simulink model "hrg_wa_v8_calibrated"  (R2025a)
settings: Solver=ode4  StartTime=0.0  StopTime=wl_stop  FixedStep=wl_Tp  RelTol=1e-3
PostLoadFcn:
  | addpath(fileparts(fileparts(get_param('hrg_wa_v8_calibrated','FileName')))); w8_setup(getVariable(get_param('hrg_wa_v8_calibrated','ModelWorkspace'),'v8_saved_configuration'));
model workspace (MAT data in the model file):
  v7_saved_configuration.stage = 5
  v7_saved_configuration.name = 'hrg_wa_v8_calibrated'
  v7_saved_configuration.head.sourceProfile = 'C:\Users\11725\Desktop\HRG_WA\HRG_WA_Digital_ASIC_MATLAB_v4_6_5_FRP_validation_fix\HRG_WA\config\head_default.json'
  v7_saved_configuration.head.measurementStatus = 'assumed, not a measured head'
  v7_saved_configuration.head.f0 = 5000
  v7_saved_configuration.head.Q = 2000000
  v7_saved_configuration.head.bryan = 0.277
  v7_saved_configuration.head.gamma = 0.00785398163397
  v7_saved_configuration.head.dgamma = 0
  v7_saved_configuration.head.dampingAxis = 0.296705972839
  v7_saved_configuration.head.splitHz = 0
  v7_saved_configuration.head.stiffnessAxis = 0.715584993318
  v7_saved_configuration.head.detuningHz = 0
  v7_saved_configuration.head.duffingHz = 0
  v7_saved_configuration.head.temperatureCoeff = -1.8e-05
  v7_saved_configuration.head.referenceTemperature = 25
  v7_saved_configuration.head.detect = [1.012  0; 0  0.989]
  v7_saved_configuration.head.detectPhase = [0; 0]
  v7_saved_configuration.head.drive = [1  0; 0  1]
  v7_saved_configuration.head.detectCubic = 0
  v7_saved_configuration.head.iqBits = 0
  v7_saved_configuration.head.iqFullScale = 2
  v7_saved_configuration.head.energyTarget = 1
  v7_saved_configuration.head.initialEnergy = 1
  v7_saved_configuration.head.initialTheta = 0.13962634016
  v7_saved_configuration.head.initialQuadRatio = 0
  v7_saved_configuration.head.energyKp = 4.02123859659
  v7_saved_configuration.head.energyKi = 12.6330936334
  v7_saved_configuration.head.quadKp = 6.03185789489
  v7_saved_configuration.head.quadKi = 28.4244606751
  v7_saved_configuration.head.pllKp = 1.28
  v7_saved_configuration.head.pllKi = 4.02123859659
  v7_saved_configuration.head.energyLimit = 20
  v7_saved_configuration.head.quadLimit = 2
  v7_saved_configuration.head.pllLimitHz = 2
  v7_saved_configuration.head.antiWindup = 5
  v7_saved_configuration.head.loopEnable = 1
  v7_saved_configuration.head.Ts = 0.001
  v7_saved_configuration.head.rateTau = 0.00353677651315
  v7_saved_configuration.head.energyThreshold = 0.02
  v7_saved_configuration.head.angleThreshold = 0.01
  v7_saved_configuration.head.duration = 12
  v7_saved_configuration.head.omega = 1.3962634016
  v7_saved_configuration.head.virtualRate = 0
  v7_saved_configuration.head.temperature = 25
  v7_saved_configuration.head.fullStep = 2e-06
  v7_saved_configuration.fsAdc = 40000
  v7_saved_configuration.fsPlant = 800000
  v7_saved_configuration.duration = 2
  v7_saved_configuration.seed = 20261021
  v7_saved_configuration.massKg = 1e-06
  v7_saved_configuration.displacementM = 4e-07
  v7_saved_configuration.gapM = 5e-06
  v7_saved_configuration.c0F = 1e-12
  v7_saved_configuration.cfF = 1e-12
  v7_saved_configuration.rfOhm = 1000000000
  v7_saved_configuration.biasV = 10
  v7_saved_configuration.cvBandwidthHz = 30000
  v7_saved_configuration.pgaBandwidthHz = 30000
  v7_saved_configuration.pgaGain = 1
  v7_saved_configuration.cvEnVrtHz = 1e-08
  v7_saved_configuration.cvInArtHz = 1e-14
  v7_saved_configuration.temperatureK = 298.15
  v7_saved_configuration.pgaNoiseVrtHz = 1e-08
  v7_saved_configuration.afeOffsetV = [0; 0]
  v7_saved_configuration.afeLimitV = 1.8
  v7_saved_configuration.adcBits = 18
  v7_saved_configuration.adcFsV = 2
  v7_saved_configuration.adcOffsetV = [0; 0]
  v7_saved_configuration.adcGain = [1; 1]
  v7_saved_configuration.adcInlCubic = 0
  v7_saved_configuration.jitterRmsS = 2e-09
  v7_saved_configuration.channelSkewS = 0
  v7_saved_configuration.adcDelay = 1
  v7_saved_configuration.adcArchitecture = 'nyquist'
  v7_saved_configuration.cicStages = 3
  v7_saved_configuration.fir = [0.111111111111 0.222222222222 0.333333333333 0.222222222222 0.111111111111]
  v7_saved_configuration.dacBits = 16
  v7_saved_configuration.dacFsV = 2
  v7_saved_configuration.dacDelay = 1
  v7_saved_configuration.dacInlCubic = 0
  v7_saved_configuration.dacArchitecture = 'nyquist'
  v7_saved_configuration.driveNPerV = 1e-07
  v7_saved_configuration.driverBandwidthHz = 50000
  v7_saved_configuration.driverGain = [1.018; 0.982]
  v7_saved_configuration.driverSlewVPerS = 200000
  v7_saved_configuration.driverNoiseVrtHz = 2e-08
  v7_saved_configuration.driverLimitV = 1.8
  v7_saved_configuration.feedthroughF = 0
  v7_saved_configuration.pipelineCtrl = 3
  v7_saved_configuration.iqFractionBits = 22
  v7_saved_configuration.controlFractionBits = 22
  v7_saved_configuration.antiAliasHz = 18000
  v7_saved_configuration.noiseEnable = 0
  v7_saved_configuration.circuitEnable = 1
  v7_saved_configuration.kalman = 1
  v7_saved_configuration.online = 0
  v7_saved_configuration.frp = 0
  v7_saved_configuration.calibrationPermit = 0
  v7_saved_configuration.frpSequence = 0
  v7_saved_configuration.frpFreeze = 0
  v7_saved_configuration.frpTheta = [0; 0; 0; 0; 0; 0; 0; 0; 0]
  v7_saved_configuration.matrixApply = 0
  v7_saved_configuration.compensationApply = 0
  v7_saved_configuration.temperatureCompensate = 0
  v7_saved_configuration.temperatureBiasCoefficients = [0; 0; 0]
  v7_saved_configuration.zeroRateCertified = 0
  v7_saved_configuration.virtualRate = 0
  v7_saved_configuration.inputRate = 1.3962634016
  v7_saved_configuration.inputFrequencyHz = 0
  v7_saved_configuration.inputRateAmplitude = 0
  v7_saved_configuration.temperatureC = 25
  v7_saved_configuration.temperatureRampCPerS = 0
  v7_saved_configuration.observers = 1
  v7_saved_configuration.spectra = 1
  v7_saved_configuration.maxLogPoints = 1600001
  v7_saved_configuration.sdmLeak = 0.9999
  v7_saved_configuration.sdmReferenceV = 2
  v7_saved_configuration.tdmEnable = 0
  v7_saved_configuration.knownPhaseCalibrationRad = 0
  v7_saved_configuration.virtualGainCalibration = 1
  v7_saved_configuration.learnStartS = 0.25
  v7_saved_configuration.measurementStatus = 'unmeasured research assumptions; replace with measured head and interface data'
  v7_saved_configuration.scope = 'Behavioral circuit interfaces, not transistor or bit-true RTL signoff'
  v7_saved_configuration.v7.schemaVersion = 1
  v7_saved_configuration.v7.status = 'unmeasured research assumptions; replace with measured head and interface data'
  v7_saved_configuration.v7.mechanicalProfile = 'HRG_WA_Digital_ASIC_MATLAB_v4_6_5_FRP_validation_fix/HRG_WA/config/head_default.json'
  v7_saved_configuration.v7.headSimulation.Ts = 0.001
  v7_saved_configuration.v7.headSimulation.initialEnergy = 1
  v7_saved_configuration.v7.headSimulation.initialQuadRatio = 0
  v7_saved_configuration.v7.headSimulation.rateTau = 0.00353677651315
  v7_saved_configuration.v7.circuit.fsAdc = 40000
  v7_saved_configuration.v7.circuit.massKg = 1e-06
  v7_saved_configuration.v7.circuit.displacementM = 1e-07
  v7_saved_configuration.v7.circuit.gapM = 5e-06
  v7_saved_configuration.v7.circuit.c0F = 1e-12
  v7_saved_configuration.v7.circuit.biasV = 10
  v7_saved_configuration.v7.circuit.cvBandwidthHz = 30000
  v7_saved_configuration.v7.circuit.pgaBandwidthHz = 30000
  v7_saved_configuration.v7.circuit.cvEnVrtHz = 1e-08
  v7_saved_configuration.v7.circuit.cvInArtHz = 1e-14
  v7_saved_configuration.v7.circuit.temperatureK = 298.15
  v7_saved_configuration.v7.circuit.pgaNoiseVrtHz = 1e-08
  v7_saved_configuration.v7.circuit.afeOffsetV = [0; 0]
  v7_saved_configuration.v7.circuit.afeLimitV = 1.8
  v7_saved_configuration.v7.circuit.adcBits = 18
  v7_saved_configuration.v7.circuit.adcFsV = 2
  v7_saved_configuration.v7.circuit.adcOffsetV = [0; 0]
  v7_saved_configuration.v7.circuit.adcGain = [1; 1]
  v7_saved_configuration.v7.circuit.adcInlCubic = 0
  v7_saved_configuration.v7.circuit.jitterRmsS = 2e-09
  v7_saved_configuration.v7.circuit.channelSkewS = 0
  v7_saved_configuration.v7.circuit.adcDelay = 1
  v7_saved_configuration.v7.circuit.adcArchitecture = 'nyquist'
  v7_saved_configuration.v7.circuit.cicStages = 3
  v7_saved_configuration.v7.circuit.fir = [0.111111111111; 0.222222222222; 0.333333333333; 0.222222222222; 0.111111111111]
  v7_saved_configuration.v7.circuit.dacBits = 16
  v7_saved_configuration.v7.circuit.dacFsV = 2
  v7_saved_configuration.v7.circuit.dacDelay = 1
  v7_saved_configuration.v7.circuit.dacInlCubic = 0
  v7_saved_configuration.v7.circuit.dacArchitecture = 'nyquist'
  v7_saved_configuration.v7.circuit.driveNPerV = 1e-07
  v7_saved_configuration.v7.circuit.driverBandwidthHz = 50000
  v7_saved_configuration.v7.circuit.driverGain = [1; 1]
  v7_saved_configuration.v7.circuit.driverSlewVPerS = 200000
  v7_saved_configuration.v7.circuit.driverNoiseVrtHz = 2e-08
  v7_saved_configuration.v7.circuit.driverLimitV = 1.8
  v7_saved_configuration.v7.circuit.feedthroughF = 0
  v7_saved_configuration.v7.circuit.pipelineCtrl = 3
  v7_saved_configuration.v7.circuit.iqFractionBits = 22
  v7_saved_configuration.v7.circuit.controlFractionBits = 22
  v7_saved_configuration.v7.circuit.antiAliasHz = 18000
  v7_saved_configuration.v7.fsPlant = 800000
  v7_saved_configuration.v7.duration = 2
  v7_saved_configuration.v7.readoutMode = 'charge'
  v7_saved_configuration.v7.charge.rfOhm = 1000000000
  v7_saved_configuration.v7.charge.cfF = 1e-12
  v7_saved_configuration.v7.charge.pgaGain = 1
  v7_saved_configuration.v7.tia.rfOhm = 1000000
  v7_saved_configuration.v7.tia.cfF = 1e-12
  v7_saved_configuration.v7.tia.pgaGain = 31.8309886184
  v7_saved_configuration.v7.loopNaturalHz = [0.8; 1.2; 0.8]
  v7_saved_configuration.v7.dampingRatio = 0.8
  v7_saved_configuration.v7.controlMode = 'PI'
  v7_saved_configuration.v7.resonantGain = [0.4; 1.2; 0]
  v7_saved_configuration.v7.resonantLeakRadS = 0.04
  v7_saved_configuration.v7.resonantMinimumRadS = 0.15
  v7_saved_configuration.v7.resonantMaximumRadS = 25
  v7_saved_configuration.v7.frequencyEstimateTauS = 0.1
  v7_saved_configuration.v7.slewPerS = [500; 100; 100]
  v7_saved_configuration.v7.startupEnable = 1
  v7_saved_configuration.v7.startupAmplitudePerS = 4
  v7_saved_configuration.v7.startupSwitchEnergy = 0.25
  v7_saved_configuration.v7.startupTimeoutS = 1.5
  v7_saved_configuration.v7.startupDirectionRad = 0
  v7_saved_configuration.v7.tdmMode = 'continuous'
  v7_saved_configuration.v7.slotCycles = [1; 1; 2; 1]
  v7_saved_configuration.v7.readBlankCycles = 0.25
  v7_saved_configuration.v7.acquisitionTauS = 2e-06
  v7_saved_configuration.v7.unloadTauS = 2e-06
  v7_saved_configuration.v7.sampleCapF = 1e-11
  v7_saved_configuration.v7.switchChargeC = [0; 0]
  v7_saved_configuration.v7.actuationMode = 'linear'
  v7_saved_configuration.v7.driveBiasV = 10
  v7_saved_configuration.v7.electrostaticForceScale = 0.025
  v7_saved_configuration.v7.budget.angleRmsRad = 1e-06
  v7_saved_configuration.v7.budget.noiseBandwidthHz = 100
  v7_saved_configuration.v7.budget.startupTimeS = 0.1
  v7_saved_configuration.v7.profile = 'C:\Users\11725\Desktop\HRG_WA\HRG_WA_simulink\literature_v7\profile.json'
  v7_saved_configuration.v7.senseCalibration = 0.228707119333+1.04243935371i
  v7_saved_configuration.v7.driveCalibration = 0.297893136802+0.987329357138i
  v7_saved_configuration.v7.nominalGram = [0.5  0; 0  0.5]
  v7_saved_configuration.v8.schemaVersion = 1
  v7_saved_configuration.v8.status = 'research assumptions and synthetic-fixture exploration, not measured head calibration'
  v7_saved_configuration.v8.enabled = 1
  v7_saved_configuration.v8.senseInverse = [0.98814229249-5.09989730271e-17i  0+0i; 0+0i  1.0111223458+9.61174803704e-17i]
  v7_saved_configuration.v8.driveInverse = [0.98231827112  0; 0  1.0183299389]
  v7_saved_configuration.v8.cubicCoefficient = [0.0049158912; 0.0046949808]
  v7_saved_configuration.v8.maximumCalibratedAmplitude = 1.5
  v7_saved_configuration.v8.correlatedThermalNoise = 1
  v7_saved_configuration.v8.extraWarmupControlFrames = 1
  v7_saved_configuration.v8.calibrationSource = 'synthetic independent-reference fixture; w8_run_studies; not measured hardware'
  v7_saved_configuration.v8.filterWarmupS = 0.012
  v7_saved_configuration.cvEquivalentNoiseVrtHz = 3.43925280635e-07
  v8_saved_configuration.stage = 5
  v8_saved_configuration.name = 'hrg_wa_v8_calibrated'
  v8_saved_configuration.head.sourceProfile = 'C:\Users\11725\Desktop\HRG_WA\HRG_WA_Digital_ASIC_MATLAB_v4_6_5_FRP_validation_fix\HRG_WA\config\head_default.json'
  v8_saved_configuration.head.measurementStatus = 'assumed, not a measured head'
  v8_saved_configuration.head.f0 = 5000
  v8_saved_configuration.head.Q = 2000000
  v8_saved_configuration.head.bryan = 0.277
  v8_saved_configuration.head.gamma = 0.00785398163397
  v8_saved_configuration.head.dgamma = 0
  v8_saved_configuration.head.dampingAxis = 0.296705972839
  v8_saved_configuration.head.splitHz = 0
  v8_saved_configuration.head.stiffnessAxis = 0.715584993318
  v8_saved_configuration.head.detuningHz = 0
  v8_saved_configuration.head.duffingHz = 0
  v8_saved_configuration.head.temperatureCoeff = -1.8e-05
  v8_saved_configuration.head.referenceTemperature = 25
  v8_saved_configuration.head.detect = [1.012  0; 0  0.989]
  v8_saved_configuration.head.detectPhase = [0; 0]
  v8_saved_configuration.head.drive = [1  0; 0  1]
  v8_saved_configuration.head.detectCubic = 0
  v8_saved_configuration.head.iqBits = 0
  v8_saved_configuration.head.iqFullScale = 2
  v8_saved_configuration.head.energyTarget = 1
  v8_saved_configuration.head.initialEnergy = 1
  v8_saved_configuration.head.initialTheta = 0.13962634016
  v8_saved_configuration.head.initialQuadRatio = 0
  v8_saved_configuration.head.energyKp = 4.02123859659
  v8_saved_configuration.head.energyKi = 12.6330936334
  v8_saved_configuration.head.quadKp = 6.03185789489
  v8_saved_configuration.head.quadKi = 28.4244606751
  v8_saved_configuration.head.pllKp = 1.28
  v8_saved_configuration.head.pllKi = 4.02123859659
  v8_saved_configuration.head.energyLimit = 20
  v8_saved_configuration.head.quadLimit = 2
  v8_saved_configuration.head.pllLimitHz = 2
  v8_saved_configuration.head.antiWindup = 5
  v8_saved_configuration.head.loopEnable = 1
  v8_saved_configuration.head.Ts = 0.001
  v8_saved_configuration.head.rateTau = 0.00353677651315
  v8_saved_configuration.head.energyThreshold = 0.02
  v8_saved_configuration.head.angleThreshold = 0.01
  v8_saved_configuration.head.duration = 12
  v8_saved_configuration.head.omega = 1.3962634016
  v8_saved_configuration.head.virtualRate = 0
  v8_saved_configuration.head.temperature = 25
  v8_saved_configuration.head.fullStep = 2e-06
  v8_saved_configuration.fsAdc = 40000
  v8_saved_configuration.fsPlant = 800000
  v8_saved_configuration.duration = 2
  v8_saved_configuration.seed = 20261021
  v8_saved_configuration.massKg = 1e-06
  v8_saved_configuration.displacementM = 4e-07
  v8_saved_configuration.gapM = 5e-06
  v8_saved_configuration.c0F = 1e-12
  v8_saved_configuration.cfF = 1e-12
  v8_saved_configuration.rfOhm = 1000000000
  v8_saved_configuration.biasV = 10
  v8_saved_configuration.cvBandwidthHz = 30000
  v8_saved_configuration.pgaBandwidthHz = 30000
  v8_saved_configuration.pgaGain = 1
  v8_saved_configuration.cvEnVrtHz = 1e-08
  v8_saved_configuration.cvInArtHz = 1e-14
  v8_saved_configuration.temperatureK = 298.15
  v8_saved_configuration.pgaNoiseVrtHz = 1e-08
  v8_saved_configuration.afeOffsetV = [0; 0]
  v8_saved_configuration.afeLimitV = 1.8
  v8_saved_configuration.adcBits = 18
  v8_saved_configuration.adcFsV = 2
  v8_saved_configuration.adcOffsetV = [0; 0]
  v8_saved_configuration.adcGain = [1; 1]
  v8_saved_configuration.adcInlCubic = 0
  v8_saved_configuration.jitterRmsS = 2e-09
  v8_saved_configuration.channelSkewS = 0
  v8_saved_configuration.adcDelay = 1
  v8_saved_configuration.adcArchitecture = 'nyquist'
  v8_saved_configuration.cicStages = 3
  v8_saved_configuration.fir = [0.111111111111 0.222222222222 0.333333333333 0.222222222222 0.111111111111]
  v8_saved_configuration.dacBits = 16
  v8_saved_configuration.dacFsV = 2
  v8_saved_configuration.dacDelay = 1
  v8_saved_configuration.dacInlCubic = 0
  v8_saved_configuration.dacArchitecture = 'nyquist'
  v8_saved_configuration.driveNPerV = 1e-07
  v8_saved_configuration.driverBandwidthHz = 50000
  v8_saved_configuration.driverGain = [1.018; 0.982]
  v8_saved_configuration.driverSlewVPerS = 200000
  v8_saved_configuration.driverNoiseVrtHz = 2e-08
  v8_saved_configuration.driverLimitV = 1.8
  v8_saved_configuration.feedthroughF = 0
  v8_saved_configuration.pipelineCtrl = 3
  v8_saved_configuration.iqFractionBits = 22
  v8_saved_configuration.controlFractionBits = 22
  v8_saved_configuration.antiAliasHz = 18000
  v8_saved_configuration.noiseEnable = 0
  v8_saved_configuration.circuitEnable = 1
  v8_saved_configuration.kalman = 1
  v8_saved_configuration.online = 0
  v8_saved_configuration.frp = 0
  v8_saved_configuration.calibrationPermit = 0
  v8_saved_configuration.frpSequence = 0
  v8_saved_configuration.frpFreeze = 0
  v8_saved_configuration.frpTheta = [0; 0; 0; 0; 0; 0; 0; 0; 0]
  v8_saved_configuration.matrixApply = 0
  v8_saved_configuration.compensationApply = 0
  v8_saved_configuration.temperatureCompensate = 0
  v8_saved_configuration.temperatureBiasCoefficients = [0; 0; 0]
  v8_saved_configuration.zeroRateCertified = 0
  v8_saved_configuration.virtualRate = 0
  v8_saved_configuration.inputRate = 1.3962634016
  v8_saved_configuration.inputFrequencyHz = 0
  v8_saved_configuration.inputRateAmplitude = 0
  v8_saved_configuration.temperatureC = 25
  v8_saved_configuration.temperatureRampCPerS = 0
  v8_saved_configuration.observers = 1
  v8_saved_configuration.spectra = 1
  v8_saved_configuration.maxLogPoints = 1600001
  v8_saved_configuration.sdmLeak = 0.9999
  v8_saved_configuration.sdmReferenceV = 2
  v8_saved_configuration.tdmEnable = 0
  v8_saved_configuration.knownPhaseCalibrationRad = 0
  v8_saved_configuration.virtualGainCalibration = 1
  v8_saved_configuration.learnStartS = 0.25
  v8_saved_configuration.measurementStatus = 'unmeasured research assumptions; replace with measured head and interface data'
  v8_saved_configuration.scope = 'Behavioral circuit interfaces, not transistor or bit-true RTL signoff'
  v8_saved_configuration.v7.schemaVersion = 1
  v8_saved_configuration.v7.status = 'unmeasured research assumptions; replace with measured head and interface data'
  v8_saved_configuration.v7.mechanicalProfile = 'HRG_WA_Digital_ASIC_MATLAB_v4_6_5_FRP_validation_fix/HRG_WA/config/head_default.json'
  v8_saved_configuration.v7.headSimulation.Ts = 0.001
  v8_saved_configuration.v7.headSimulation.initialEnergy = 1
  v8_saved_configuration.v7.headSimulation.initialQuadRatio = 0
  v8_saved_configuration.v7.headSimulation.rateTau = 0.00353677651315
  v8_saved_configuration.v7.circuit.fsAdc = 40000
  v8_saved_configuration.v7.circuit.massKg = 1e-06
  v8_saved_configuration.v7.circuit.displacementM = 1e-07
  v8_saved_configuration.v7.circuit.gapM = 5e-06
  v8_saved_configuration.v7.circuit.c0F = 1e-12
  v8_saved_configuration.v7.circuit.biasV = 10
  v8_saved_configuration.v7.circuit.cvBandwidthHz = 30000
  v8_saved_configuration.v7.circuit.pgaBandwidthHz = 30000
  v8_saved_configuration.v7.circuit.cvEnVrtHz = 1e-08
  v8_saved_configuration.v7.circuit.cvInArtHz = 1e-14
  v8_saved_configuration.v7.circuit.temperatureK = 298.15
  v8_saved_configuration.v7.circuit.pgaNoiseVrtHz = 1e-08
  v8_saved_configuration.v7.circuit.afeOffsetV = [0; 0]
  v8_saved_configuration.v7.circuit.afeLimitV = 1.8
  v8_saved_configuration.v7.circuit.adcBits = 18
  v8_saved_configuration.v7.circuit.adcFsV = 2
  v8_saved_configuration.v7.circuit.adcOffsetV = [0; 0]
  v8_saved_configuration.v7.circuit.adcGain = [1; 1]
  v8_saved_configuration.v7.circuit.adcInlCubic = 0
  v8_saved_configuration.v7.circuit.jitterRmsS = 2e-09
  v8_saved_configuration.v7.circuit.channelSkewS = 0
  v8_saved_configuration.v7.circuit.adcDelay = 1
  v8_saved_configuration.v7.circuit.adcArchitecture = 'nyquist'
  v8_saved_configuration.v7.circuit.cicStages = 3
  v8_saved_configuration.v7.circuit.fir = [0.111111111111; 0.222222222222; 0.333333333333; 0.222222222222; 0.111111111111]
  v8_saved_configuration.v7.circuit.dacBits = 16
  v8_saved_configuration.v7.circuit.dacFsV = 2
  v8_saved_configuration.v7.circuit.dacDelay = 1
  v8_saved_configuration.v7.circuit.dacInlCubic = 0
  v8_saved_configuration.v7.circuit.dacArchitecture = 'nyquist'
  v8_saved_configuration.v7.circuit.driveNPerV = 1e-07
  v8_saved_configuration.v7.circuit.driverBandwidthHz = 50000
  v8_saved_configuration.v7.circuit.driverGain = [1; 1]
  v8_saved_configuration.v7.circuit.driverSlewVPerS = 200000
  v8_saved_configuration.v7.circuit.driverNoiseVrtHz = 2e-08
  v8_saved_configuration.v7.circuit.driverLimitV = 1.8
  v8_saved_configuration.v7.circuit.feedthroughF = 0
  v8_saved_configuration.v7.circuit.pipelineCtrl = 3
  v8_saved_configuration.v7.circuit.iqFractionBits = 22
  v8_saved_configuration.v7.circuit.controlFractionBits = 22
  v8_saved_configuration.v7.circuit.antiAliasHz = 18000
  v8_saved_configuration.v7.fsPlant = 800000
  v8_saved_configuration.v7.duration = 2
  v8_saved_configuration.v7.readoutMode = 'charge'
  v8_saved_configuration.v7.charge.rfOhm = 1000000000
  v8_saved_configuration.v7.charge.cfF = 1e-12
  v8_saved_configuration.v7.charge.pgaGain = 1
  v8_saved_configuration.v7.tia.rfOhm = 1000000
  v8_saved_configuration.v7.tia.cfF = 1e-12
  v8_saved_configuration.v7.tia.pgaGain = 31.8309886184
  v8_saved_configuration.v7.loopNaturalHz = [0.8; 1.2; 0.8]
  v8_saved_configuration.v7.dampingRatio = 0.8
  v8_saved_configuration.v7.controlMode = 'PI'
  v8_saved_configuration.v7.resonantGain = [0.4; 1.2; 0]
  v8_saved_configuration.v7.resonantLeakRadS = 0.04
  v8_saved_configuration.v7.resonantMinimumRadS = 0.15
  v8_saved_configuration.v7.resonantMaximumRadS = 25
  v8_saved_configuration.v7.frequencyEstimateTauS = 0.1
  v8_saved_configuration.v7.slewPerS = [500; 100; 100]
  v8_saved_configuration.v7.startupEnable = 1
  v8_saved_configuration.v7.startupAmplitudePerS = 4
  v8_saved_configuration.v7.startupSwitchEnergy = 0.25
  v8_saved_configuration.v7.startupTimeoutS = 1.5
  v8_saved_configuration.v7.startupDirectionRad = 0
  v8_saved_configuration.v7.tdmMode = 'continuous'
  v8_saved_configuration.v7.slotCycles = [1; 1; 2; 1]
  v8_saved_configuration.v7.readBlankCycles = 0.25
  v8_saved_configuration.v7.acquisitionTauS = 2e-06
  v8_saved_configuration.v7.unloadTauS = 2e-06
  v8_saved_configuration.v7.sampleCapF = 1e-11
  v8_saved_configuration.v7.switchChargeC = [0; 0]
  v8_saved_configuration.v7.actuationMode = 'linear'
  v8_saved_configuration.v7.driveBiasV = 10
  v8_saved_configuration.v7.electrostaticForceScale = 0.025
  v8_saved_configuration.v7.budget.angleRmsRad = 1e-06
  v8_saved_configuration.v7.budget.noiseBandwidthHz = 100
  v8_saved_configuration.v7.budget.startupTimeS = 0.1
  v8_saved_configuration.v7.profile = 'C:\Users\11725\Desktop\HRG_WA\HRG_WA_simulink\literature_v7\profile.json'
  v8_saved_configuration.v7.senseCalibration = 0.228707119333+1.04243935371i
  v8_saved_configuration.v7.driveCalibration = 0.297893136802+0.987329357138i
  v8_saved_configuration.v7.nominalGram = [0.5  0; 0  0.5]
  v8_saved_configuration.v8.schemaVersion = 1
  v8_saved_configuration.v8.status = 'research assumptions and synthetic-fixture exploration, not measured head calibration'
  v8_saved_configuration.v8.enabled = 1
  v8_saved_configuration.v8.senseInverse = [0.98814229249-5.09989730271e-17i  0+0i; 0+0i  1.0111223458+9.61174803704e-17i]
  v8_saved_configuration.v8.driveInverse = [0.98231827112  0; 0  1.0183299389]
  v8_saved_configuration.v8.cubicCoefficient = [0.0049158912; 0.0046949808]
  v8_saved_configuration.v8.maximumCalibratedAmplitude = 1.5
  v8_saved_configuration.v8.correlatedThermalNoise = 1
  v8_saved_configuration.v8.extraWarmupControlFrames = 1
  v8_saved_configuration.v8.calibrationSource = 'synthetic independent-reference fixture; w8_run_studies; not measured hardware'
  v8_saved_configuration.v8.filterWarmupS = 0.012
  v8_saved_configuration.cvEquivalentNoiseVrtHz = 3.43925280635e-07
  wl_saved_configuration.stage = 5
  wl_saved_configuration.name = 'hrg_wa_v8_calibrated'
  wl_saved_configuration.head.sourceProfile = 'C:\Users\11725\Desktop\HRG_WA\HRG_WA_Digital_ASIC_MATLAB_v4_6_5_FRP_validation_fix\HRG_WA\config\head_default.json'
  wl_saved_configuration.head.measurementStatus = 'assumed, not a measured head'
  wl_saved_configuration.head.f0 = 5000
  wl_saved_configuration.head.Q = 2000000
  wl_saved_configuration.head.bryan = 0.277
  wl_saved_configuration.head.gamma = 0.00785398163397
  wl_saved_configuration.head.dgamma = 0
  wl_saved_configuration.head.dampingAxis = 0.296705972839
  wl_saved_configuration.head.splitHz = 0
  wl_saved_configuration.head.stiffnessAxis = 0.715584993318
  wl_saved_configuration.head.detuningHz = 0
  wl_saved_configuration.head.duffingHz = 0
  wl_saved_configuration.head.temperatureCoeff = -1.8e-05
  wl_saved_configuration.head.referenceTemperature = 25
  wl_saved_configuration.head.detect = [1.012  0; 0  0.989]
  wl_saved_configuration.head.detectPhase = [0; 0]
  wl_saved_configuration.head.drive = [1  0; 0  1]
  wl_saved_configuration.head.detectCubic = 0
  wl_saved_configuration.head.iqBits = 0
  wl_saved_configuration.head.iqFullScale = 2
  wl_saved_configuration.head.energyTarget = 1
  wl_saved_configuration.head.initialEnergy = 1
  wl_saved_configuration.head.initialTheta = 0.13962634016
  wl_saved_configuration.head.initialQuadRatio = 0
  wl_saved_configuration.head.energyKp = 4.02123859659
  wl_saved_configuration.head.energyKi = 12.6330936334
  wl_saved_configuration.head.quadKp = 6.03185789489
  wl_saved_configuration.head.quadKi = 28.4244606751
  wl_saved_configuration.head.pllKp = 1.28
  wl_saved_configuration.head.pllKi = 4.02123859659
  wl_saved_configuration.head.energyLimit = 20
  wl_saved_configuration.head.quadLimit = 2
  wl_saved_configuration.head.pllLimitHz = 2
  wl_saved_configuration.head.antiWindup = 5
  wl_saved_configuration.head.loopEnable = 1
  wl_saved_configuration.head.Ts = 0.001
  wl_saved_configuration.head.rateTau = 0.00353677651315
  wl_saved_configuration.head.energyThreshold = 0.02
  wl_saved_configuration.head.angleThreshold = 0.01
  wl_saved_configuration.head.duration = 12
  wl_saved_configuration.head.omega = 1.3962634016
  wl_saved_configuration.head.virtualRate = 0
  wl_saved_configuration.head.temperature = 25
  wl_saved_configuration.head.fullStep = 2e-06
  wl_saved_configuration.fsAdc = 40000
  wl_saved_configuration.fsPlant = 800000
  wl_saved_configuration.duration = 2
  wl_saved_configuration.seed = 20261021
  wl_saved_configuration.massKg = 1e-06
  wl_saved_configuration.displacementM = 4e-07
  wl_saved_configuration.gapM = 5e-06
  wl_saved_configuration.c0F = 1e-12
  wl_saved_configuration.cfF = 1e-12
  wl_saved_configuration.rfOhm = 1000000000
  wl_saved_configuration.biasV = 10
  wl_saved_configuration.cvBandwidthHz = 30000
  wl_saved_configuration.pgaBandwidthHz = 30000
  wl_saved_configuration.pgaGain = 1
  wl_saved_configuration.cvEnVrtHz = 1e-08
  wl_saved_configuration.cvInArtHz = 1e-14
  wl_saved_configuration.temperatureK = 298.15
  wl_saved_configuration.pgaNoiseVrtHz = 1e-08
  wl_saved_configuration.afeOffsetV = [0; 0]
  wl_saved_configuration.afeLimitV = 1.8
  wl_saved_configuration.adcBits = 18
  wl_saved_configuration.adcFsV = 2
  wl_saved_configuration.adcOffsetV = [0; 0]
  wl_saved_configuration.adcGain = [1; 1]
  wl_saved_configuration.adcInlCubic = 0
  wl_saved_configuration.jitterRmsS = 2e-09
  wl_saved_configuration.channelSkewS = 0
  wl_saved_configuration.adcDelay = 1
  wl_saved_configuration.adcArchitecture = 'nyquist'
  wl_saved_configuration.cicStages = 3
  wl_saved_configuration.fir = [0.111111111111 0.222222222222 0.333333333333 0.222222222222 0.111111111111]
  wl_saved_configuration.dacBits = 16
  wl_saved_configuration.dacFsV = 2
  wl_saved_configuration.dacDelay = 1
  wl_saved_configuration.dacInlCubic = 0
  wl_saved_configuration.dacArchitecture = 'nyquist'
  wl_saved_configuration.driveNPerV = 1e-07
  wl_saved_configuration.driverBandwidthHz = 50000
  wl_saved_configuration.driverGain = [1.018; 0.982]
  wl_saved_configuration.driverSlewVPerS = 200000
  wl_saved_configuration.driverNoiseVrtHz = 2e-08
  wl_saved_configuration.driverLimitV = 1.8
  wl_saved_configuration.feedthroughF = 0
  wl_saved_configuration.pipelineCtrl = 3
  wl_saved_configuration.iqFractionBits = 22
  wl_saved_configuration.controlFractionBits = 22
  wl_saved_configuration.antiAliasHz = 18000
  wl_saved_configuration.noiseEnable = 0
  wl_saved_configuration.circuitEnable = 1
  wl_saved_configuration.kalman = 1
  wl_saved_configuration.online = 0
  wl_saved_configuration.frp = 0
  wl_saved_configuration.calibrationPermit = 0
  wl_saved_configuration.frpSequence = 0
  wl_saved_configuration.frpFreeze = 0
  wl_saved_configuration.frpTheta = [0; 0; 0; 0; 0; 0; 0; 0; 0]
  wl_saved_configuration.matrixApply = 0
  wl_saved_configuration.compensationApply = 0
  wl_saved_configuration.temperatureCompensate = 0
  wl_saved_configuration.temperatureBiasCoefficients = [0; 0; 0]
  wl_saved_configuration.zeroRateCertified = 0
  wl_saved_configuration.virtualRate = 0
  wl_saved_configuration.inputRate = 1.3962634016
  wl_saved_configuration.inputFrequencyHz = 0
  wl_saved_configuration.inputRateAmplitude = 0
  wl_saved_configuration.temperatureC = 25
  wl_saved_configuration.temperatureRampCPerS = 0
  wl_saved_configuration.observers = 1
  wl_saved_configuration.spectra = 1
  wl_saved_configuration.maxLogPoints = 1600001
  wl_saved_configuration.sdmLeak = 0.9999
  wl_saved_configuration.sdmReferenceV = 2
  wl_saved_configuration.tdmEnable = 0
  wl_saved_configuration.knownPhaseCalibrationRad = 0
  wl_saved_configuration.virtualGainCalibration = 1
  wl_saved_configuration.learnStartS = 0.25
  wl_saved_configuration.measurementStatus = 'unmeasured research assumptions; replace with measured head and interface data'
  wl_saved_configuration.scope = 'Behavioral circuit interfaces, not transistor or bit-true RTL signoff'
  wl_saved_configuration.v7.schemaVersion = 1
  wl_saved_configuration.v7.status = 'unmeasured research assumptions; replace with measured head and interface data'
  wl_saved_configuration.v7.mechanicalProfile = 'HRG_WA_Digital_ASIC_MATLAB_v4_6_5_FRP_validation_fix/HRG_WA/config/head_default.json'
  wl_saved_configuration.v7.headSimulation.Ts = 0.001
  wl_saved_configuration.v7.headSimulation.initialEnergy = 1
  wl_saved_configuration.v7.headSimulation.initialQuadRatio = 0
  wl_saved_configuration.v7.headSimulation.rateTau = 0.00353677651315
  wl_saved_configuration.v7.circuit.fsAdc = 40000
  wl_saved_configuration.v7.circuit.massKg = 1e-06
  wl_saved_configuration.v7.circuit.displacementM = 1e-07
  wl_saved_configuration.v7.circuit.gapM = 5e-06
  wl_saved_configuration.v7.circuit.c0F = 1e-12
  wl_saved_configuration.v7.circuit.biasV = 10
  wl_saved_configuration.v7.circuit.cvBandwidthHz = 30000
  wl_saved_configuration.v7.circuit.pgaBandwidthHz = 30000
  wl_saved_configuration.v7.circuit.cvEnVrtHz = 1e-08
  wl_saved_configuration.v7.circuit.cvInArtHz = 1e-14
  wl_saved_configuration.v7.circuit.temperatureK = 298.15
  wl_saved_configuration.v7.circuit.pgaNoiseVrtHz = 1e-08
  wl_saved_configuration.v7.circuit.afeOffsetV = [0; 0]
  wl_saved_configuration.v7.circuit.afeLimitV = 1.8
  wl_saved_configuration.v7.circuit.adcBits = 18
  wl_saved_configuration.v7.circuit.adcFsV = 2
  wl_saved_configuration.v7.circuit.adcOffsetV = [0; 0]
  wl_saved_configuration.v7.circuit.adcGain = [1; 1]
  wl_saved_configuration.v7.circuit.adcInlCubic = 0
  wl_saved_configuration.v7.circuit.jitterRmsS = 2e-09
  wl_saved_configuration.v7.circuit.channelSkewS = 0
  wl_saved_configuration.v7.circuit.adcDelay = 1
  wl_saved_configuration.v7.circuit.adcArchitecture = 'nyquist'
  wl_saved_configuration.v7.circuit.cicStages = 3
  wl_saved_configuration.v7.circuit.fir = [0.111111111111; 0.222222222222; 0.333333333333; 0.222222222222; 0.111111111111]
  wl_saved_configuration.v7.circuit.dacBits = 16
  wl_saved_configuration.v7.circuit.dacFsV = 2
  wl_saved_configuration.v7.circuit.dacDelay = 1
  wl_saved_configuration.v7.circuit.dacInlCubic = 0
  wl_saved_configuration.v7.circuit.dacArchitecture = 'nyquist'
  wl_saved_configuration.v7.circuit.driveNPerV = 1e-07
  wl_saved_configuration.v7.circuit.driverBandwidthHz = 50000
  wl_saved_configuration.v7.circuit.driverGain = [1; 1]
  wl_saved_configuration.v7.circuit.driverSlewVPerS = 200000
  wl_saved_configuration.v7.circuit.driverNoiseVrtHz = 2e-08
  wl_saved_configuration.v7.circuit.driverLimitV = 1.8
  wl_saved_configuration.v7.circuit.feedthroughF = 0
  wl_saved_configuration.v7.circuit.pipelineCtrl = 3
  wl_saved_configuration.v7.circuit.iqFractionBits = 22
  wl_saved_configuration.v7.circuit.controlFractionBits = 22
  wl_saved_configuration.v7.circuit.antiAliasHz = 18000
  wl_saved_configuration.v7.fsPlant = 800000
  wl_saved_configuration.v7.duration = 2
  wl_saved_configuration.v7.readoutMode = 'charge'
  wl_saved_configuration.v7.charge.rfOhm = 1000000000
  wl_saved_configuration.v7.charge.cfF = 1e-12
  wl_saved_configuration.v7.charge.pgaGain = 1
  wl_saved_configuration.v7.tia.rfOhm = 1000000
  wl_saved_configuration.v7.tia.cfF = 1e-12
  wl_saved_configuration.v7.tia.pgaGain = 31.8309886184
  wl_saved_configuration.v7.loopNaturalHz = [0.8; 1.2; 0.8]
  wl_saved_configuration.v7.dampingRatio = 0.8
  wl_saved_configuration.v7.controlMode = 'PI'
  wl_saved_configuration.v7.resonantGain = [0.4; 1.2; 0]
  wl_saved_configuration.v7.resonantLeakRadS = 0.04
  wl_saved_configuration.v7.resonantMinimumRadS = 0.15
  wl_saved_configuration.v7.resonantMaximumRadS = 25
  wl_saved_configuration.v7.frequencyEstimateTauS = 0.1
  wl_saved_configuration.v7.slewPerS = [500; 100; 100]
  wl_saved_configuration.v7.startupEnable = 1
  wl_saved_configuration.v7.startupAmplitudePerS = 4
  wl_saved_configuration.v7.startupSwitchEnergy = 0.25
  wl_saved_configuration.v7.startupTimeoutS = 1.5
  wl_saved_configuration.v7.startupDirectionRad = 0
  wl_saved_configuration.v7.tdmMode = 'continuous'
  wl_saved_configuration.v7.slotCycles = [1; 1; 2; 1]
  wl_saved_configuration.v7.readBlankCycles = 0.25
  wl_saved_configuration.v7.acquisitionTauS = 2e-06
  wl_saved_configuration.v7.unloadTauS = 2e-06
  wl_saved_configuration.v7.sampleCapF = 1e-11
  wl_saved_configuration.v7.switchChargeC = [0; 0]
  wl_saved_configuration.v7.actuationMode = 'linear'
  wl_saved_configuration.v7.driveBiasV = 10
  wl_saved_configuration.v7.electrostaticForceScale = 0.025
  wl_saved_configuration.v7.budget.angleRmsRad = 1e-06
  wl_saved_configuration.v7.budget.noiseBandwidthHz = 100
  wl_saved_configuration.v7.budget.startupTimeS = 0.1
  wl_saved_configuration.v7.profile = 'C:\Users\11725\Desktop\HRG_WA\HRG_WA_simulink\literature_v7\profile.json'
  wl_saved_configuration.v7.senseCalibration = 0.228707119333+1.04243935371i
  wl_saved_configuration.v7.driveCalibration = 0.297893136802+0.987329357138i
  wl_saved_configuration.v7.nominalGram = [0.5  0; 0  0.5]
  wl_saved_configuration.v8.schemaVersion = 1
  wl_saved_configuration.v8.status = 'research assumptions and synthetic-fixture exploration, not measured head calibration'
  wl_saved_configuration.v8.enabled = 1
  wl_saved_configuration.v8.senseInverse = [0.98814229249-5.09989730271e-17i  0+0i; 0+0i  1.0111223458+9.61174803704e-17i]
  wl_saved_configuration.v8.driveInverse = [0.98231827112  0; 0  1.0183299389]
  wl_saved_configuration.v8.cubicCoefficient = [0.0049158912; 0.0046949808]
  wl_saved_configuration.v8.maximumCalibratedAmplitude = 1.5
  wl_saved_configuration.v8.correlatedThermalNoise = 1
  wl_saved_configuration.v8.extraWarmupControlFrames = 1
  wl_saved_configuration.v8.calibrationSource = 'synthetic independent-reference fixture; w8_run_studies; not measured hardware'
  wl_saved_configuration.v8.filterWarmupS = 0.012
  wl_saved_configuration.cvEquivalentNoiseVrtHz = 3.43925722091e-07
undefined symbols (not defined in the file): w7_force, w7_mix, w8_control_tick, w8_feedback_gate, w8_iq, wl_adc_transfer, wl_boxcar, wl_brownVariance, wl_c, wl_capacitance, wl_cvGain, wl_cvNoiseVariance, wl_cvTau, wl_D, wl_detectGain, wl_driverNoiseVariance, wl_fir, wl_hToV, wl_input, wl_J, wl_jitterVariance, wl_K, wl_modulate, wl_pgaNoiseVariance, wl_q0, wl_quantize, wl_R, wl_Ta, wl_Tc, wl_Tp, wl_v0
settings Model: Creator=11725  LastModifiedBy=11725
settings DataIOCC: SaveOutput=off
settings DebuggingCC: SignalInfNanChecking=error  AlgebraicLoopMsg=error

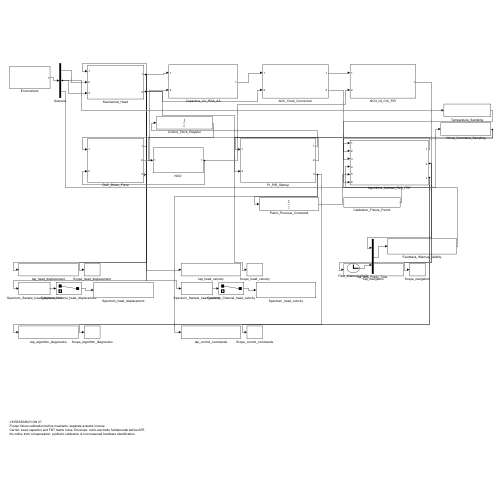
[thumbnail: Simulink's stored preview of the top-level diagram]
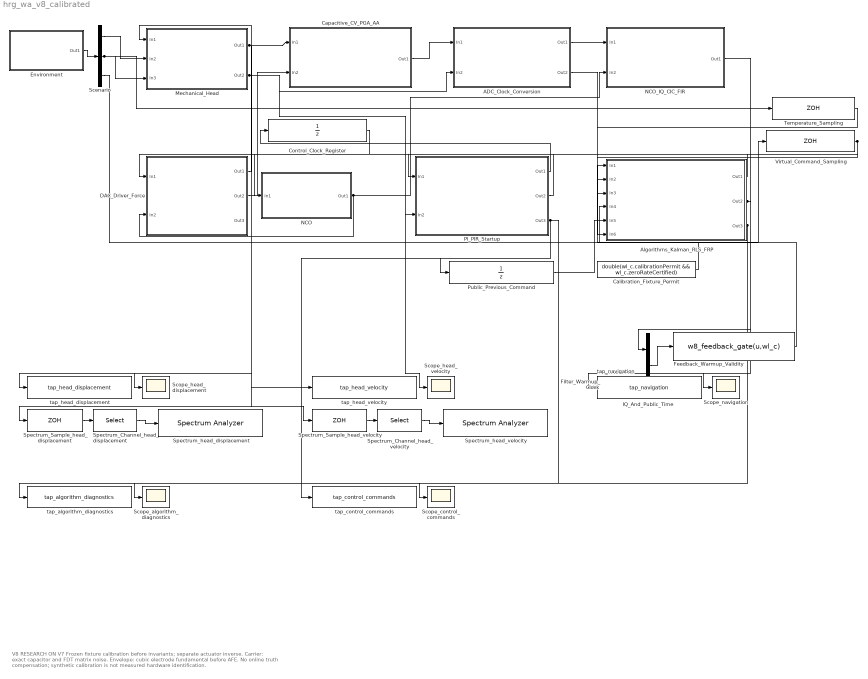
== system hrg_wa_v8_calibrated ==
  note: V8 RESEARCH ON V7
      | Frozen fixture calibration before invariants; separate actuator inverse.
      | Carrier: exact capacitor and FDT matrix noise. Envelope: cubic electrode fundamental before AFE.
      | No online truth compensation; synthetic calibration is not measured hardware identification.
  ADC_Clock_Conversion : Subsystem
  Algorithms_Kalman_RLS_FRP : Subsystem
  Calibration_Fixture_Permit : Constant  Value=double(wl_c.calibrationPermit && wl_c.zeroRateCertified)
  Capacitive_CV_PGA_AA : Subsystem
  Control_Clock_Register : UnitDelay  InitialCondition=zeros(4,1)  SampleTime=wl_Tc  HasFrameUpgradeWarning=on
  DAC_Driver_Force : Subsystem
  Environment : Subsystem
  Feedback_Warmup_Validity : MATLABFcn  MATLABFcn=w8_feedback_gate(u,wl_c)  OutputDimensions=4
  Filter_Warmup_Clock : Clock
  IQ_And_Public_Time : Mux  Inputs=2
  Mechanical_Head : Subsystem
  NCO : Subsystem
  NCO_IQ_CIC_FIR : Subsystem
  PI_PIR_Startup : Subsystem
  Public_Previous_Command : UnitDelay  InitialCondition=zeros(3,1)  SampleTime=wl_Tc  HasFrameUpgradeWarning=on
  Scenario : Demux  Outputs=[2 1 1]
  Scope_algorithm_diagnostics : Scope
  Scope_control_commands : Scope
  Scope_head_displacement : Scope
  Scope_head_velocity : Scope
  Scope_navigation : Scope
  Spectrum_Channel_head_displacement : Selector  InputPortWidth=2  IndexOptions=Index vector (dialog)  Indices=1  OutputSizes=1
  Spectrum_Channel_head_velocity : Selector  InputPortWidth=2  IndexOptions=Index vector (dialog)  Indices=1  OutputSizes=1
  Spectrum_Sample_head_displacement : ZeroOrderHold  SampleTime=1.2500000000000001e-06
  Spectrum_Sample_head_velocity : ZeroOrderHold  SampleTime=1.2500000000000001e-06
  Spectrum_head_displacement : SpectrumAnalyzer  SampleRateSource=Property  SampleRate=800000  RBWSource=Property  RBW=781.25  WindowInvariantSamplesPerUpdate=on  SpectrumUnits=dBFS  FullScaleSource=Property  Title=head_displacement - reference amplitude 1 [normalized displacement], first channel
      settings: OpenAtSimulationStart=off
  Spectrum_head_velocity : SpectrumAnalyzer  SampleRateSource=Property  SampleRate=800000  RBWSource=Property  RBW=781.25  WindowInvariantSamplesPerUpdate=on  SpectrumUnits=dBFS  FullScaleSource=Property  Title=head_velocity - reference amplitude 1 [normalized displacement/s], first channel
      settings: OpenAtSimulationStart=off
  Temperature_Sampling : ZeroOrderHold  SampleTime=wl_Tc
  Virtual_Command_Sampling : ZeroOrderHold  SampleTime=wl_Tc
  tap_algorithm_diagnostics : ToWorkspace  VariableName=tap_algorithm_diagnostics  SaveFormat=Timeseries  SampleTime=-1
      settings: MaxDataPoints=1600001
  tap_control_commands : ToWorkspace  VariableName=tap_control_commands  SaveFormat=Timeseries  SampleTime=-1
      settings: MaxDataPoints=1600001
  tap_head_displacement : ToWorkspace  VariableName=tap_head_displacement  SaveFormat=Timeseries  SampleTime=-1
      settings: MaxDataPoints=1600001
  tap_head_velocity : ToWorkspace  VariableName=tap_head_velocity  SaveFormat=Timeseries  SampleTime=-1
      settings: MaxDataPoints=1600001
  tap_navigation : ToWorkspace  VariableName=tap_navigation  SaveFormat=Timeseries  SampleTime=-1
      settings: MaxDataPoints=1600001
  wires:
  Environment/1(Out1) -> Scenario/1
  Scenario/1 -> Mechanical_Head/2(In2)
  Scenario/2 -> Mechanical_Head/3(In3), Temperature_Sampling/1
  DAC_Driver_Force/1(Out1) -> Mechanical_Head/1(In1)
  Mechanical_Head/1(Out1) -> Capacitive_CV_PGA_AA/1(In1), tap_head_displacement/1, Scope_head_displacement/1, Spectrum_Sample_head_displacement/1
  DAC_Driver_Force/2(Out2) -> Capacitive_CV_PGA_AA/2(In2)
  Capacitive_CV_PGA_AA/1(Out1) -> ADC_Clock_Conversion/1(In1)
  Mechanical_Head/2(Out2) -> ADC_Clock_Conversion/2(In2), tap_head_velocity/1, Scope_head_velocity/1, Spectrum_Sample_head_velocity/1
  ADC_Clock_Conversion/1(Out1) -> NCO_IQ_CIC_FIR/1(In1)
  NCO/1(Out1) -> NCO_IQ_CIC_FIR/2(In2), DAC_Driver_Force/2(In2)
  Scenario/3 -> Virtual_Command_Sampling/1
  Temperature_Sampling/1 -> Algorithms_Kalman_RLS_FRP/2(In2)
  Virtual_Command_Sampling/1 -> Algorithms_Kalman_RLS_FRP/3(In3), PI_PIR_Startup/2(In2)
  Calibration_Fixture_Permit/1 -> Algorithms_Kalman_RLS_FRP/4(In4)
  PI_PIR_Startup/3(Out3) -> Public_Previous_Command/1, tap_control_commands/1, Scope_control_commands/1
  Public_Previous_Command/1 -> Algorithms_Kalman_RLS_FRP/5(In5)
  Algorithms_Kalman_RLS_FRP/1(Out1) -> PI_PIR_Startup/1(In1)
  PI_PIR_Startup/2(Out2) -> NCO/1(In1)
  PI_PIR_Startup/1(Out1) -> Control_Clock_Register/1
  Control_Clock_Register/1 -> DAC_Driver_Force/1(In1)
  ADC_Clock_Conversion/2(Out2) -> Algorithms_Kalman_RLS_FRP/6(In6)
  Spectrum_Sample_head_displacement/1 -> Spectrum_Channel_head_displacement/1
  Spectrum_Channel_head_displacement/1 -> Spectrum_head_displacement/1
  Spectrum_Sample_head_velocity/1 -> Spectrum_Channel_head_velocity/1
  Spectrum_Channel_head_velocity/1 -> Spectrum_head_velocity/1
  Algorithms_Kalman_RLS_FRP/2(Out2) -> tap_navigation/1, Scope_navigation/1
  Algorithms_Kalman_RLS_FRP/3(Out3) -> tap_algorithm_diagnostics/1, Scope_algorithm_diagnostics/1
  NCO_IQ_CIC_FIR/1(Out1) -> IQ_And_Public_Time/1
  Filter_Warmup_Clock/1 -> IQ_And_Public_Time/2
  IQ_And_Public_Time/1 -> Feedback_Warmup_Validity/1
  Feedback_Warmup_Validity/1 -> Algorithms_Kalman_RLS_FRP/1(In1)

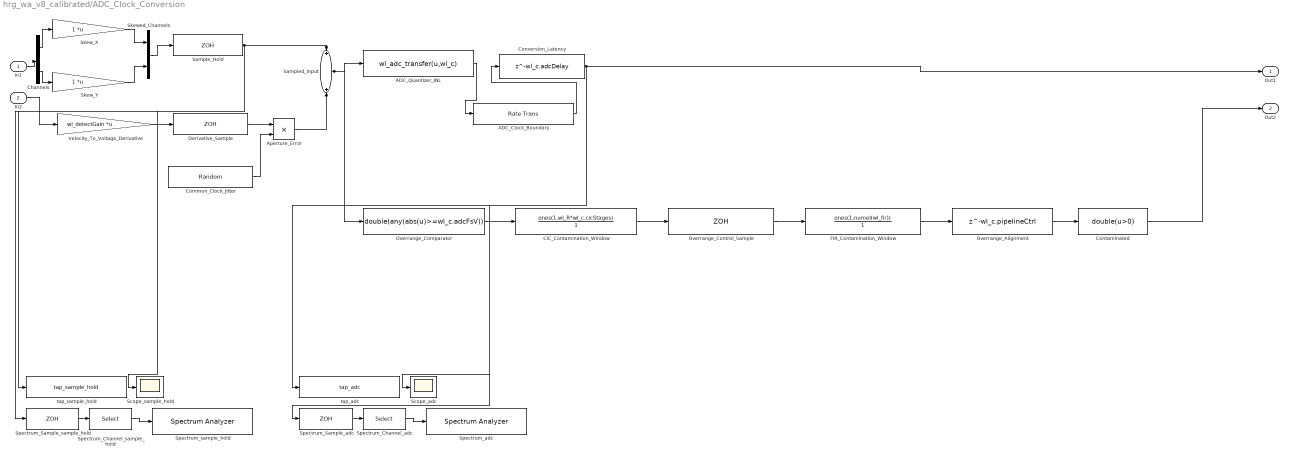
== system hrg_wa_v8_calibrated/ADC_Clock_Conversion ==
  In1 : Inport
  In2 : Inport  Port=2
  ADC_Clock_Boundary : RateTransition  Integrity=off  Deterministic=off  OutPortSampleTime=wl_Ta
  ADC_Quantizer_INL : MATLABFcn  MATLABFcn=wl_adc_transfer(u,wl_c)  OutputDimensions=2
  Aperture_Error : Product
  CIC_Contamination_Window : DiscreteFilter  Numerator=ones(1,wl_R*wl_c.cicStages)  Denominator=1  SampleTime=wl_Ta
  Channels : Demux  Outputs=2
  Common_Clock_Jitter : RandomNumber  Variance=wl_jitterVariance  Seed=wl_c.seed+621  SampleTime=wl_Ta
  Contaminated : MATLABFcn  MATLABFcn=double(u>0)  OutputDimensions=1
  Conversion_Latency : Delay  DelayLength=wl_c.adcDelay  InitialCondition=0  SampleTime=wl_Ta
  Derivative_Sample : ZeroOrderHold  SampleTime=wl_Ta
  FIR_Contamination_Window : DiscreteFilter  Numerator=ones(1,numel(wl_fir))  Denominator=1  SampleTime=wl_Tc
  Overrange_Alignment : Delay  DelayLength=wl_c.pipelineCtrl  InitialCondition=0  SampleTime=wl_Tc
  Overrange_Comparator : MATLABFcn  MATLABFcn=double(any(abs(u)>=wl_c.adcFsV))  OutputDimensions=1
  Overrange_Control_Sample : ZeroOrderHold  SampleTime=wl_Tc
  Sample_Hold : ZeroOrderHold  SampleTime=wl_Ta
  Sampled_Input : Sum
  Scope_adc : Scope
  Scope_sample_hold : Scope
  Skew_X : Gain  Multiplication=Matrix(K*u)
  Skew_Y : Gain  Multiplication=Matrix(K*u)
  Skewed_Channels : Mux  Inputs=2
  Spectrum_Channel_adc : Selector  InputPortWidth=2  IndexOptions=Index vector (dialog)  Indices=1  OutputSizes=1
  Spectrum_Channel_sample_hold : Selector  InputPortWidth=2  IndexOptions=Index vector (dialog)  Indices=1  OutputSizes=1
  Spectrum_Sample_adc : ZeroOrderHold  SampleTime=2.5000000000000001e-05
  Spectrum_Sample_sample_hold : ZeroOrderHold  SampleTime=2.5000000000000001e-05
  Spectrum_adc : SpectrumAnalyzer  SampleRateSource=Property  SampleRate=40000  RBWSource=Property  RBW=39.0625  WindowInvariantSamplesPerUpdate=on  SpectrumUnits=dBV  Title=adc - voltage power spectrum (first channel)
      settings: OpenAtSimulationStart=off
  Spectrum_sample_hold : SpectrumAnalyzer  SampleRateSource=Property  SampleRate=40000  RBWSource=Property  RBW=39.0625  WindowInvariantSamplesPerUpdate=on  SpectrumUnits=dBV  Title=sample_hold - voltage power spectrum (first channel)
      settings: OpenAtSimulationStart=off
  Velocity_To_Voltage_Derivative : Gain  Gain=wl_detectGain  Multiplication=Matrix(K*u)
  tap_adc : ToWorkspace  VariableName=tap_adc  SaveFormat=Timeseries  SampleTime=-1
      settings: MaxDataPoints=1600001
  tap_sample_hold : ToWorkspace  VariableName=tap_sample_hold  SaveFormat=Timeseries  SampleTime=-1
      settings: MaxDataPoints=1600001
  Out1 : Outport
  Out2 : Outport  Port=2
  wires:
  In1/1 -> Channels/1
  Channels/1 -> Skew_X/1
  Channels/2 -> Skew_Y/1
  Skew_X/1 -> Skewed_Channels/1
  Skew_Y/1 -> Skewed_Channels/2
  Skewed_Channels/1 -> Sample_Hold/1
  In2/1 -> Velocity_To_Voltage_Derivative/1
  Velocity_To_Voltage_Derivative/1 -> Derivative_Sample/1
  Derivative_Sample/1 -> Aperture_Error/1
  Common_Clock_Jitter/1 -> Aperture_Error/2
  Sample_Hold/1 -> Sampled_Input/1, tap_sample_hold/1, Scope_sample_hold/1, Spectrum_Sample_sample_hold/1
  Aperture_Error/1 -> Sampled_Input/2
  Sampled_Input/1 -> ADC_Quantizer_INL/1, Overrange_Comparator/1
  ADC_Quantizer_INL/1 -> ADC_Clock_Boundary/1
  ADC_Clock_Boundary/1 -> Conversion_Latency/1
  Conversion_Latency/1 -> Out1/1, tap_adc/1, Scope_adc/1, Spectrum_Sample_adc/1
  Overrange_Comparator/1 -> CIC_Contamination_Window/1
  CIC_Contamination_Window/1 -> Overrange_Control_Sample/1
  Overrange_Control_Sample/1 -> FIR_Contamination_Window/1
  FIR_Contamination_Window/1 -> Overrange_Alignment/1
  Overrange_Alignment/1 -> Contaminated/1
  Contaminated/1 -> Out2/1
  Spectrum_Sample_sample_hold/1 -> Spectrum_Channel_sample_hold/1
  Spectrum_Channel_sample_hold/1 -> Spectrum_sample_hold/1
  Spectrum_Sample_adc/1 -> Spectrum_Channel_adc/1
  Spectrum_Channel_adc/1 -> Spectrum_adc/1

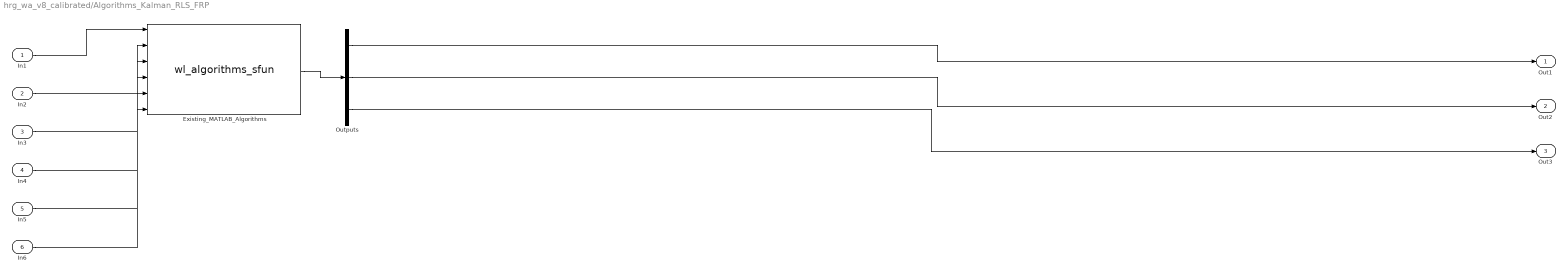
== system hrg_wa_v8_calibrated/Algorithms_Kalman_RLS_FRP ==
  In1 : Inport
  In2 : Inport  Port=2
  In3 : Inport  Port=3
  In4 : Inport  Port=4
  In5 : Inport  Port=5
  In6 : Inport  Port=6
  Existing_MATLAB_Algorithms : M-S-Function  FunctionName=wl_algorithms_sfun  Parameters=wl_c
  Outputs : Demux  Outputs=[10 4 21]
  Out1 : Outport
  Out2 : Outport  Port=2
  Out3 : Outport  Port=3
  wires:
  In1/1 -> Existing_MATLAB_Algorithms/1
  In2/1 -> Existing_MATLAB_Algorithms/2
  In3/1 -> Existing_MATLAB_Algorithms/3
  In4/1 -> Existing_MATLAB_Algorithms/4
  In5/1 -> Existing_MATLAB_Algorithms/5
  In6/1 -> Existing_MATLAB_Algorithms/6
  Existing_MATLAB_Algorithms/1 -> Outputs/1
  Outputs/1 -> Out1/1
  Outputs/2 -> Out2/1
  Outputs/3 -> Out3/1

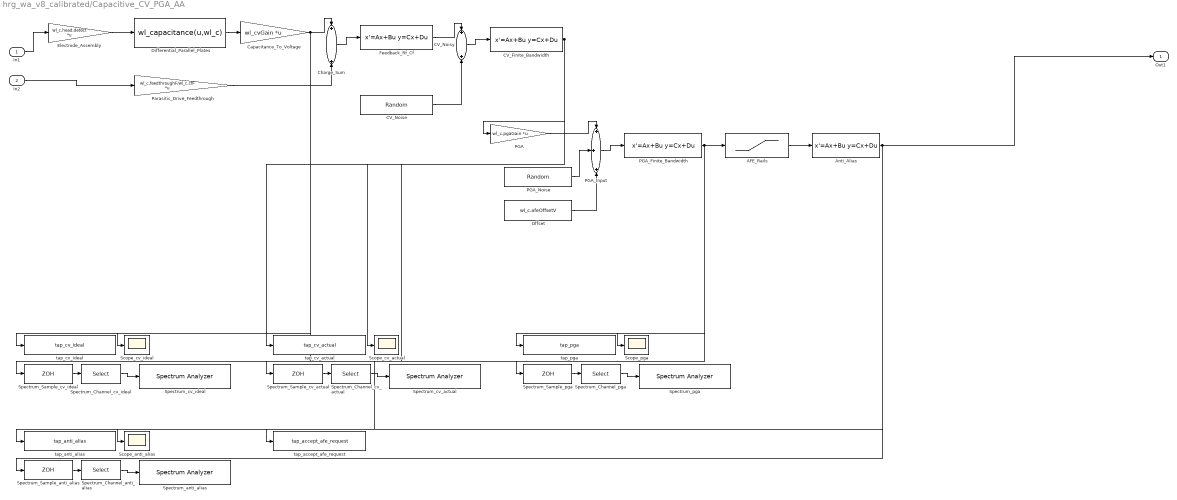
== system hrg_wa_v8_calibrated/Capacitive_CV_PGA_AA ==
  In1 : Inport
  In2 : Inport  Port=2
  AFE_Rails : Saturate  UpperLimit=wl_c.afeLimitV  LowerLimit=-wl_c.afeLimitV
  Anti_Alias : StateSpace  A=-2*pi*wl_c.antiAliasHz*eye(2)  B=2*pi*wl_c.antiAliasHz*eye(2)  C=eye(2)  D=zeros(2)  InitialCondition=0
  CV_Finite_Bandwidth : StateSpace  A=-2*pi*wl_c.cvBandwidthHz*eye(2)  B=2*pi*wl_c.cvBandwidthHz*eye(2)  C=eye(2)  D=zeros(2)  InitialCondition=0
  CV_Noise : RandomNumber  Mean=[0;0]  Variance=wl_cvNoiseVariance*[1;1]  Seed=[wl_c.seed+601;wl_c.seed+602]  SampleTime=wl_Tp
  CV_Noisy : Sum
  Capacitance_To_Voltage : Gain  Gain=wl_cvGain  Multiplication=Matrix(K*u)
  Charge_Sum : Sum
  Differential_Parallel_Plates : MATLABFcn  MATLABFcn=wl_capacitance(u,wl_c)  OutputDimensions=2
  Electrode_Assembly : Gain  Gain=wl_c.head.detect  Multiplication=Matrix(K*u)
  Feedback_Rf_Cf : StateSpace  A=-eye(2)/wl_cvTau  B=eye(2)/wl_cvTau  C=-eye(2)  D=eye(2)  InitialCondition=0
  Offset : Constant  Value=wl_c.afeOffsetV
  PGA : Gain  Gain=wl_c.pgaGain  Multiplication=Matrix(K*u)
  PGA_Finite_Bandwidth : StateSpace  A=-2*pi*wl_c.pgaBandwidthHz*eye(2)  B=2*pi*wl_c.pgaBandwidthHz*eye(2)  C=eye(2)  D=zeros(2)  InitialCondition=0
  PGA_Input : Sum  Inputs=+++
  PGA_Noise : RandomNumber  Mean=[0;0]  Variance=wl_pgaNoiseVariance*[1;1]  Seed=[wl_c.seed+611;wl_c.seed+612]  SampleTime=wl_Tp
  Parasitic_Drive_Feedthrough : Gain  Gain=wl_c.feedthroughF/wl_c.cfF  Multiplication=Matrix(K*u)
  Scope_anti_alias : Scope
  Scope_cv_actual : Scope
  Scope_cv_ideal : Scope
  Scope_pga : Scope
  Spectrum_Channel_anti_alias : Selector  InputPortWidth=2  IndexOptions=Index vector (dialog)  Indices=1  OutputSizes=1
  Spectrum_Channel_cv_actual : Selector  InputPortWidth=2  IndexOptions=Index vector (dialog)  Indices=1  OutputSizes=1
  Spectrum_Channel_cv_ideal : Selector  InputPortWidth=2  IndexOptions=Index vector (dialog)  Indices=1  OutputSizes=1
  Spectrum_Channel_pga : Selector  InputPortWidth=2  IndexOptions=Index vector (dialog)  Indices=1  OutputSizes=1
  Spectrum_Sample_anti_alias : ZeroOrderHold  SampleTime=1.2500000000000001e-06
  Spectrum_Sample_cv_actual : ZeroOrderHold  SampleTime=1.2500000000000001e-06
  Spectrum_Sample_cv_ideal : ZeroOrderHold  SampleTime=1.2500000000000001e-06
  Spectrum_Sample_pga : ZeroOrderHold  SampleTime=1.2500000000000001e-06
  Spectrum_anti_alias : SpectrumAnalyzer  SampleRateSource=Property  SampleRate=800000  RBWSource=Property  RBW=781.25  WindowInvariantSamplesPerUpdate=on  SpectrumUnits=dBV  Title=anti_alias - voltage power spectrum (first channel)
      settings: OpenAtSimulationStart=off
  Spectrum_cv_actual : SpectrumAnalyzer  SampleRateSource=Property  SampleRate=800000  RBWSource=Property  RBW=781.25  WindowInvariantSamplesPerUpdate=on  SpectrumUnits=dBV  Title=cv_actual - voltage power spectrum (first channel)
      settings: OpenAtSimulationStart=off
  Spectrum_cv_ideal : SpectrumAnalyzer  SampleRateSource=Property  SampleRate=800000  RBWSource=Property  RBW=781.25  WindowInvariantSamplesPerUpdate=on  SpectrumUnits=dBV  Title=cv_ideal - voltage power spectrum (first channel)
      settings: OpenAtSimulationStart=off
  Spectrum_pga : SpectrumAnalyzer  SampleRateSource=Property  SampleRate=800000  RBWSource=Property  RBW=781.25  WindowInvariantSamplesPerUpdate=on  SpectrumUnits=dBV  Title=pga - voltage power spectrum (first channel)
      settings: OpenAtSimulationStart=off
  tap_accept_afe_request : ToWorkspace  VariableName=tap_accept_afe_request  SaveFormat=Timeseries  SampleTime=-1
      settings: MaxDataPoints=1600001
  tap_anti_alias : ToWorkspace  VariableName=tap_anti_alias  SaveFormat=Timeseries  SampleTime=-1
      settings: MaxDataPoints=1600001
  tap_cv_actual : ToWorkspace  VariableName=tap_cv_actual  SaveFormat=Timeseries  SampleTime=-1
      settings: MaxDataPoints=1600001
  tap_cv_ideal : ToWorkspace  VariableName=tap_cv_ideal  SaveFormat=Timeseries  SampleTime=-1
      settings: MaxDataPoints=1600001
  tap_pga : ToWorkspace  VariableName=tap_pga  SaveFormat=Timeseries  SampleTime=-1
      settings: MaxDataPoints=1600001
  Out1 : Outport
  wires:
  In1/1 -> Electrode_Assembly/1
  Electrode_Assembly/1 -> Differential_Parallel_Plates/1
  Differential_Parallel_Plates/1 -> Capacitance_To_Voltage/1
  In2/1 -> Parasitic_Drive_Feedthrough/1
  Capacitance_To_Voltage/1 -> Charge_Sum/1, tap_cv_ideal/1, Scope_cv_ideal/1, Spectrum_Sample_cv_ideal/1
  Parasitic_Drive_Feedthrough/1 -> Charge_Sum/2
  Charge_Sum/1 -> Feedback_Rf_Cf/1
  Feedback_Rf_Cf/1 -> CV_Noisy/1
  CV_Noise/1 -> CV_Noisy/2
  CV_Noisy/1 -> CV_Finite_Bandwidth/1
  CV_Finite_Bandwidth/1 -> PGA/1, tap_cv_actual/1, Scope_cv_actual/1, Spectrum_Sample_cv_actual/1
  PGA/1 -> PGA_Input/1
  PGA_Noise/1 -> PGA_Input/2
  Offset/1 -> PGA_Input/3
  PGA_Input/1 -> PGA_Finite_Bandwidth/1
  PGA_Finite_Bandwidth/1 -> AFE_Rails/1, tap_pga/1, Scope_pga/1, Spectrum_Sample_pga/1, tap_accept_afe_request/1
  AFE_Rails/1 -> Anti_Alias/1
  Anti_Alias/1 -> Out1/1, tap_anti_alias/1, Scope_anti_alias/1, Spectrum_Sample_anti_alias/1
  Spectrum_Sample_cv_ideal/1 -> Spectrum_Channel_cv_ideal/1
  Spectrum_Channel_cv_ideal/1 -> Spectrum_cv_ideal/1
  Spectrum_Sample_cv_actual/1 -> Spectrum_Channel_cv_actual/1
  Spectrum_Channel_cv_actual/1 -> Spectrum_cv_actual/1
  Spectrum_Sample_pga/1 -> Spectrum_Channel_pga/1
  Spectrum_Channel_pga/1 -> Spectrum_pga/1
  Spectrum_Sample_anti_alias/1 -> Spectrum_Channel_anti_alias/1
  Spectrum_Channel_anti_alias/1 -> Spectrum_anti_alias/1

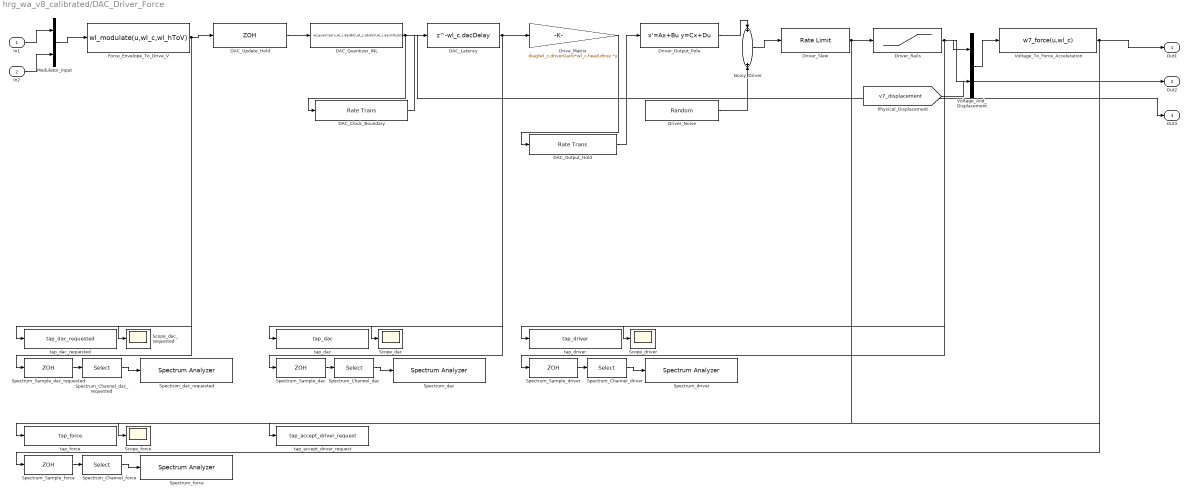
== system hrg_wa_v8_calibrated/DAC_Driver_Force ==
  In1 : Inport
  In2 : Inport  Port=2
  DAC_Clock_Boundary : RateTransition  Integrity=off  Deterministic=off  OutPortSampleTime=wl_Ta
  DAC_Latency : Delay  DelayLength=wl_c.dacDelay  InitialCondition=0  SampleTime=wl_Ta
  DAC_Output_Hold : RateTransition  Integrity=off  Deterministic=off  OutPortSampleTime=0
  DAC_Quantizer_INL : MATLABFcn  MATLABFcn=wl_quantize(u,wl_c.dacBits,wl_c.dacFsV,wl_c.dacInlCubic)  OutputDimensions=2
  DAC_Update_Hold : ZeroOrderHold  SampleTime=wl_Ta
  Drive_Matrix : Gain  Gain=diag(wl_c.driverGain)*wl_c.head.drive  Multiplication=Matrix(K*u)
  Driver_Noise : RandomNumber  Mean=[0;0]  Variance=wl_driverNoiseVariance*[1;1]  Seed=[wl_c.seed+631;wl_c.seed+632]  SampleTime=wl_Tp
  Driver_Output_Pole : StateSpace  A=-2*pi*wl_c.driverBandwidthHz*eye(2)  B=2*pi*wl_c.driverBandwidthHz*eye(2)  C=eye(2)  D=zeros(2)  InitialCondition=0
  Driver_Rails : Saturate  UpperLimit=wl_c.driverLimitV  LowerLimit=-wl_c.driverLimitV
  Driver_Slew : RateLimiter  RisingSlewLimit=wl_c.driverSlewVPerS  FallingSlewLimit=-wl_c.driverSlewVPerS  SampleTimeMode=inherited
  Force_Envelope_To_Drive_V : MATLABFcn  MATLABFcn=wl_modulate(u,wl_c,wl_hToV)  OutputDimensions=2
  Modulator_Input : Mux  Inputs=2
  Noisy_Driver : Sum
  Scope_dac : Scope
  Scope_dac_requested : Scope
  Scope_driver : Scope
  Scope_force : Scope
  Spectrum_Channel_dac : Selector  InputPortWidth=2  IndexOptions=Index vector (dialog)  Indices=1  OutputSizes=1
  Spectrum_Channel_dac_requested : Selector  InputPortWidth=2  IndexOptions=Index vector (dialog)  Indices=1  OutputSizes=1
  Spectrum_Channel_driver : Selector  InputPortWidth=2  IndexOptions=Index vector (dialog)  Indices=1  OutputSizes=1
  Spectrum_Channel_force : Selector  InputPortWidth=2  IndexOptions=Index vector (dialog)  Indices=1  OutputSizes=1
  Spectrum_Sample_dac : ZeroOrderHold  SampleTime=2.5000000000000001e-05
  Spectrum_Sample_dac_requested : ZeroOrderHold  SampleTime=1.2500000000000001e-06
  Spectrum_Sample_driver : ZeroOrderHold  SampleTime=1.2500000000000001e-06
  Spectrum_Sample_force : ZeroOrderHold  SampleTime=1.2500000000000001e-06
  Spectrum_dac : SpectrumAnalyzer  SampleRateSource=Property  SampleRate=40000  RBWSource=Property  RBW=39.0625  WindowInvariantSamplesPerUpdate=on  SpectrumUnits=dBV  Title=dac - voltage power spectrum (first channel)
      settings: OpenAtSimulationStart=off
  Spectrum_dac_requested : SpectrumAnalyzer  SampleRateSource=Property  SampleRate=800000  RBWSource=Property  RBW=781.25  WindowInvariantSamplesPerUpdate=on  SpectrumUnits=dBV  Title=dac_requested - voltage power spectrum (first channel)
      settings: OpenAtSimulationStart=off
  Spectrum_driver : SpectrumAnalyzer  SampleRateSource=Property  SampleRate=800000  RBWSource=Property  RBW=781.25  WindowInvariantSamplesPerUpdate=on  SpectrumUnits=dBV  Title=driver - voltage power spectrum (first channel)
      settings: OpenAtSimulationStart=off
  Spectrum_force : SpectrumAnalyzer  SampleRateSource=Property  SampleRate=800000  RBWSource=Property  RBW=781.25  WindowInvariantSamplesPerUpdate=on  SpectrumUnits=dBFS  FullScaleSource=Property  Title=force - reference amplitude 1 [normalized acceleration], first channel
      settings: OpenAtSimulationStart=off
  Voltage_And_Displacement : Mux  Inputs=2
  Voltage_To_Force_Acceleration : MATLABFcn  MATLABFcn=w7_force(u,wl_c)  OutputDimensions=2
  tap_accept_driver_request : ToWorkspace  VariableName=tap_accept_driver_request  SaveFormat=Timeseries  SampleTime=-1
      settings: MaxDataPoints=1600001
  tap_dac : ToWorkspace  VariableName=tap_dac  SaveFormat=Timeseries  SampleTime=-1
      settings: MaxDataPoints=1600001
  tap_dac_requested : ToWorkspace  VariableName=tap_dac_requested  SaveFormat=Timeseries  SampleTime=-1
      settings: MaxDataPoints=1600001
  tap_driver : ToWorkspace  VariableName=tap_driver  SaveFormat=Timeseries  SampleTime=-1
      settings: MaxDataPoints=1600001
  tap_force : ToWorkspace  VariableName=tap_force  SaveFormat=Timeseries  SampleTime=-1
      settings: MaxDataPoints=1600001
  Out1 : Outport
  Out2 : Outport  Port=2
  Out3 : Outport  Port=3
  wires:
  In1/1 -> Modulator_Input/1
  In2/1 -> Modulator_Input/2
  Modulator_Input/1 -> Force_Envelope_To_Drive_V/1
  Force_Envelope_To_Drive_V/1 -> DAC_Update_Hold/1, tap_dac_requested/1, Scope_dac_requested/1, Spectrum_Sample_dac_requested/1
  DAC_Update_Hold/1 -> DAC_Quantizer_INL/1
  DAC_Quantizer_INL/1 -> DAC_Clock_Boundary/1, Out3/1
  DAC_Clock_Boundary/1 -> DAC_Latency/1
  DAC_Latency/1 -> Drive_Matrix/1, tap_dac/1, Scope_dac/1, Spectrum_Sample_dac/1
  Drive_Matrix/1 -> DAC_Output_Hold/1
  DAC_Output_Hold/1 -> Driver_Output_Pole/1
  Driver_Output_Pole/1 -> Noisy_Driver/1
  Driver_Noise/1 -> Noisy_Driver/2
  Noisy_Driver/1 -> Driver_Slew/1
  Driver_Slew/1 -> Driver_Rails/1, tap_accept_driver_request/1
  Driver_Rails/1 -> Out2/1, tap_driver/1, Scope_driver/1, Spectrum_Sample_driver/1, Voltage_And_Displacement/1
  Spectrum_Sample_dac_requested/1 -> Spectrum_Channel_dac_requested/1
  Spectrum_Channel_dac_requested/1 -> Spectrum_dac_requested/1
  Spectrum_Sample_dac/1 -> Spectrum_Channel_dac/1
  Spectrum_Channel_dac/1 -> Spectrum_dac/1
  Spectrum_Sample_driver/1 -> Spectrum_Channel_driver/1
  Spectrum_Channel_driver/1 -> Spectrum_driver/1
  Spectrum_Sample_force/1 -> Spectrum_Channel_force/1
  Spectrum_Channel_force/1 -> Spectrum_force/1
  [v7_displacement] -> Voltage_And_Displacement/2
  Voltage_And_Displacement/1 -> Voltage_To_Force_Acceleration/1
  Voltage_To_Force_Acceleration/1 -> Out1/1, tap_force/1, Scope_force/1, Spectrum_Sample_force/1

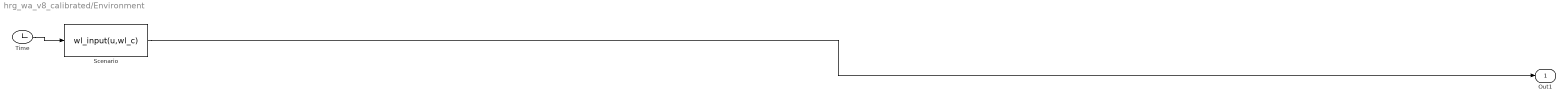
== system hrg_wa_v8_calibrated/Environment ==
  Scenario : MATLABFcn  MATLABFcn=wl_input(u,wl_c)  OutputDimensions=4
  Time : Clock
  Out1 : Outport
  wires:
  Time/1 -> Scenario/1
  Scenario/1 -> Out1/1

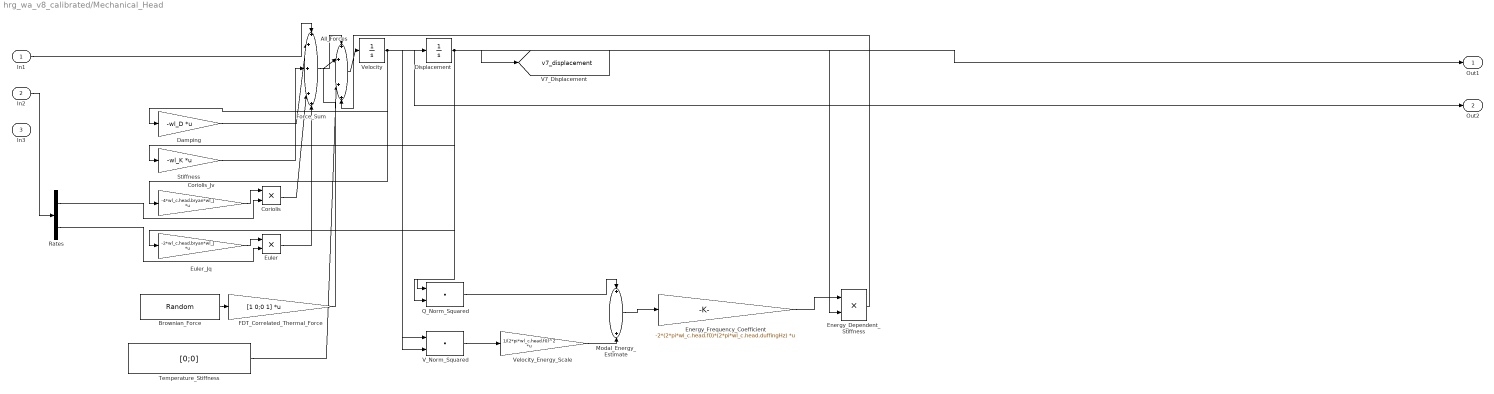
== system hrg_wa_v8_calibrated/Mechanical_Head ==
  In1 : Inport
  In2 : Inport  Port=2
  In3 : Inport  Port=3
  All_Forces : Sum  Inputs=++++
  Brownian_Force : RandomNumber  Mean=[0;0]  Variance=wl_brownVariance*[1;1]  Seed=[wl_c.seed+501;wl_c.seed+502]  SampleTime=wl_Tp
  Coriolis : Product
  Coriolis_Jv : Gain  Gain=-4*wl_c.head.bryan*wl_J  Multiplication=Matrix(K*u)
  Damping : Gain  Gain=-wl_D  Multiplication=Matrix(K*u)
  Displacement : Integrator  InitialCondition=wl_q0
  Energy_Dependent_Stiffness : Product
  Energy_Frequency_Coefficient : Gain  Gain=-2*(2*pi*wl_c.head.f0)*(2*pi*wl_c.head.duffingHz)  Multiplication=Matrix(K*u)
  Euler : Product
  Euler_Jq : Gain  Gain=-2*wl_c.head.bryan*wl_J  Multiplication=Matrix(K*u)
  FDT_Correlated_Thermal_Force : Gain  Gain=[1 0;0 1]  Multiplication=Matrix(K*u)
  Force_Sum : Sum  Inputs=+++++
  Modal_Energy_Estimate : Sum
  Q_Norm_Squared : DotProduct  OutDataTypeStr=Inherit: Inherit via internal rule
  Rates : Demux  Outputs=2
  Stiffness : Gain  Gain=-wl_K  Multiplication=Matrix(K*u)
  Temperature_Stiffness : Constant  Value=[0;0]
  V_Norm_Squared : DotProduct  OutDataTypeStr=Inherit: Inherit via internal rule
  Velocity : Integrator  InitialCondition=wl_v0
  Velocity_Energy_Scale : Gain  Gain=1/(2*pi*wl_c.head.f0)^2  Multiplication=Matrix(K*u)
  Out1 : Outport
  Out2 : Outport  Port=2
  tag scope: v7_displacement=global
  wires:
  In1/1 -> Force_Sum/1
  Velocity/1 -> Damping/1, Coriolis_Jv/1, V_Norm_Squared/1, V_Norm_Squared/2, Displacement/1, Out2/1
  Damping/1 -> Force_Sum/2
  Displacement/1 -> Stiffness/1, Euler_Jq/1, Q_Norm_Squared/1, Q_Norm_Squared/2, Energy_Dependent_Stiffness/2, Out1/1, [v7_displacement]
  Stiffness/1 -> Force_Sum/3
  In2/1 -> Rates/1
  Coriolis_Jv/1 -> Coriolis/1
  Rates/1 -> Coriolis/2
  Euler_Jq/1 -> Euler/1
  Rates/2 -> Euler/2
  Coriolis/1 -> Force_Sum/4
  Euler/1 -> Force_Sum/5
  V_Norm_Squared/1 -> Velocity_Energy_Scale/1
  Q_Norm_Squared/1 -> Modal_Energy_Estimate/1
  Velocity_Energy_Scale/1 -> Modal_Energy_Estimate/2
  Modal_Energy_Estimate/1 -> Energy_Frequency_Coefficient/1
  Energy_Frequency_Coefficient/1 -> Energy_Dependent_Stiffness/1
  Energy_Dependent_Stiffness/1 -> All_Forces/4
  Force_Sum/1 -> All_Forces/1
  Temperature_Stiffness/1 -> All_Forces/3
  All_Forces/1 -> Velocity/1
  Brownian_Force/1 -> FDT_Correlated_Thermal_Force/1
  FDT_Correlated_Thermal_Force/1 -> All_Forces/2

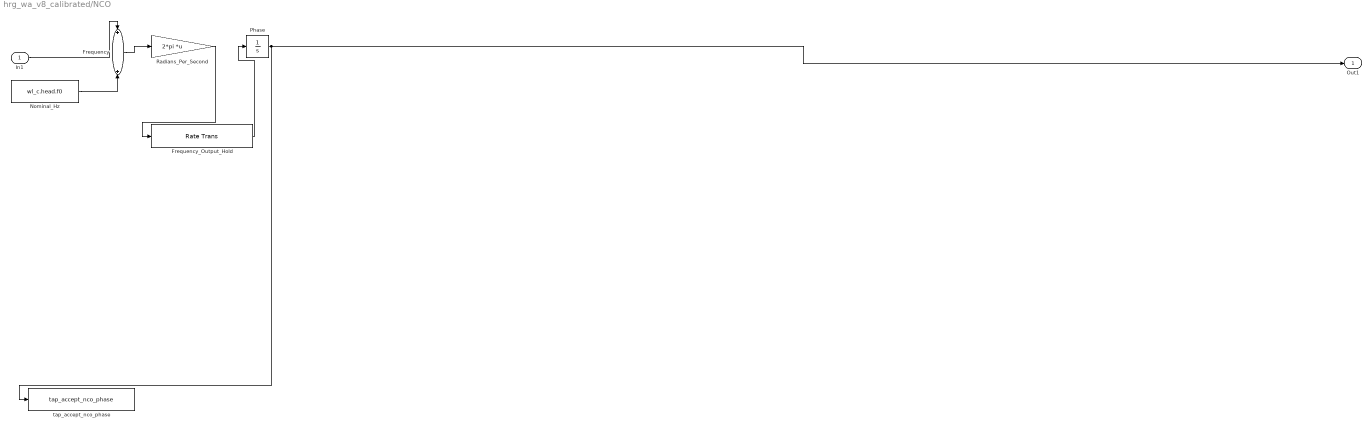
== system hrg_wa_v8_calibrated/NCO ==
  In1 : Inport
  Frequency : Sum
  Frequency_Output_Hold : RateTransition  Integrity=off  Deterministic=off  OutPortSampleTime=0
  Nominal_Hz : Constant  Value=wl_c.head.f0
  Phase : Integrator
  Radians_Per_Second : Gain  Gain=2*pi  Multiplication=Matrix(K*u)
  tap_accept_nco_phase : ToWorkspace  VariableName=tap_accept_nco_phase  SaveFormat=Timeseries  SampleTime=-1
      settings: MaxDataPoints=1600001
  Out1 : Outport
  wires:
  In1/1 -> Frequency/1
  Nominal_Hz/1 -> Frequency/2
  Frequency/1 -> Radians_Per_Second/1
  Radians_Per_Second/1 -> Frequency_Output_Hold/1
  Frequency_Output_Hold/1 -> Phase/1
  Phase/1 -> Out1/1, tap_accept_nco_phase/1

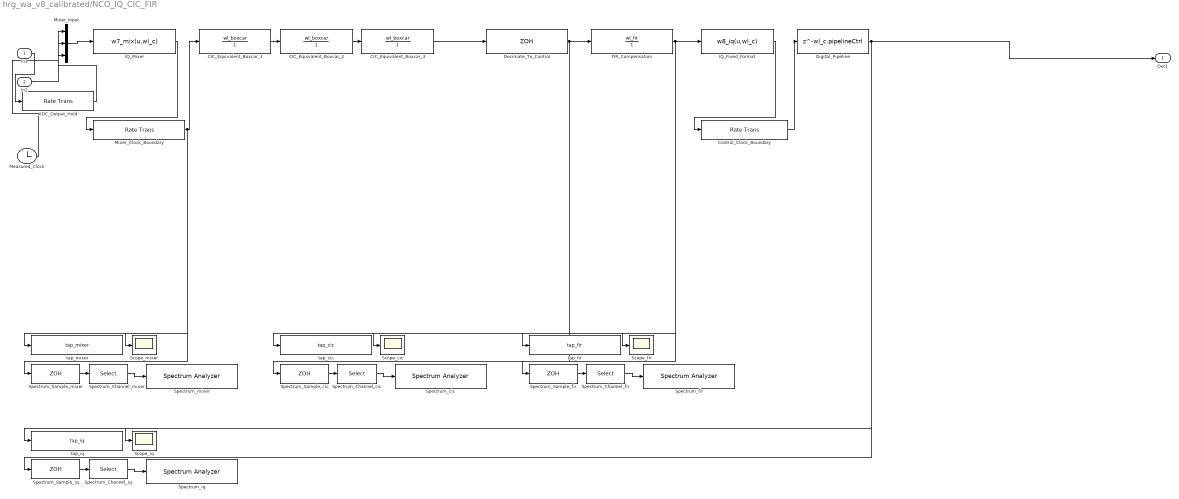
== system hrg_wa_v8_calibrated/NCO_IQ_CIC_FIR ==
  In1 : Inport
  In2 : Inport  Port=2
  ADC_Output_Hold : RateTransition  Integrity=off  Deterministic=off  OutPortSampleTime=0
  CIC_Equivalent_Boxcar_1 : DiscreteFilter  Numerator=wl_boxcar  Denominator=1  SampleTime=wl_Ta
  CIC_Equivalent_Boxcar_2 : DiscreteFilter  Numerator=wl_boxcar  Denominator=1  SampleTime=wl_Ta
  CIC_Equivalent_Boxcar_3 : DiscreteFilter  Numerator=wl_boxcar  Denominator=1  SampleTime=wl_Ta
  Control_Clock_Boundary : RateTransition  Integrity=off  Deterministic=off  OutPortSampleTime=wl_Tc
  Decimate_To_Control : ZeroOrderHold  SampleTime=wl_Tc
  Digital_Pipeline : Delay  DelayLength=wl_c.pipelineCtrl  InitialCondition=0  SampleTime=wl_Tc
  FIR_Compensation : DiscreteFilter  Numerator=wl_fir  Denominator=1  SampleTime=wl_Tc
  IQ_Fixed_Format : MATLABFcn  MATLABFcn=w8_iq(u,wl_c)  OutputDimensions=4
  IQ_Mixer : MATLABFcn  MATLABFcn=w7_mix(u,wl_c)  OutputDimensions=4
  Measured_Clock : Clock
  Mixer_Clock_Boundary : RateTransition  Integrity=off  Deterministic=off  OutPortSampleTime=wl_Ta
  Mixer_Input : Mux  Inputs=3
  Scope_cic : Scope
  Scope_fir : Scope
  Scope_iq : Scope
  Scope_mixer : Scope
  Spectrum_Channel_cic : Selector  InputPortWidth=4  IndexOptions=Index vector (dialog)  Indices=1  OutputSizes=1
  Spectrum_Channel_fir : Selector  InputPortWidth=4  IndexOptions=Index vector (dialog)  Indices=1  OutputSizes=1
  Spectrum_Channel_iq : Selector  InputPortWidth=4  IndexOptions=Index vector (dialog)  Indices=1  OutputSizes=1
  Spectrum_Channel_mixer : Selector  InputPortWidth=4  IndexOptions=Index vector (dialog)  Indices=1  OutputSizes=1
  Spectrum_Sample_cic : ZeroOrderHold  SampleTime=0.001
  Spectrum_Sample_fir : ZeroOrderHold  SampleTime=0.001
  Spectrum_Sample_iq : ZeroOrderHold  SampleTime=0.001
  Spectrum_Sample_mixer : ZeroOrderHold  SampleTime=2.5000000000000001e-05
  Spectrum_cic : SpectrumAnalyzer  SampleRateSource=Property  SampleRate=1000  RBWSource=Property  RBW=1  WindowInvariantSamplesPerUpdate=on  SpectrumUnits=dBFS  FullScaleSource=Property  Title=cic Cx: slow signal spectrum, not isolated noise; ref=1
      settings: OpenAtSimulationStart=off
  Spectrum_fir : SpectrumAnalyzer  SampleRateSource=Property  SampleRate=1000  RBWSource=Property  RBW=1  WindowInvariantSamplesPerUpdate=on  SpectrumUnits=dBFS  FullScaleSource=Property  Title=fir Cx: slow signal spectrum, not isolated noise; ref=1
      settings: OpenAtSimulationStart=off
  Spectrum_iq : SpectrumAnalyzer  SampleRateSource=Property  SampleRate=1000  RBWSource=Property  RBW=1  WindowInvariantSamplesPerUpdate=on  SpectrumUnits=dBFS  FullScaleSource=Property  Title=iq Cx: slow signal spectrum, not isolated noise; ref=1
      settings: OpenAtSimulationStart=off
  Spectrum_mixer : SpectrumAnalyzer  SampleRateSource=Property  SampleRate=40000  RBWSource=Property  RBW=39.0625  WindowInvariantSamplesPerUpdate=on  SpectrumUnits=dBFS  FullScaleSource=Property  Title=mixer Cx: slow signal spectrum, not isolated noise; ref=1
      settings: OpenAtSimulationStart=off
  tap_cic : ToWorkspace  VariableName=tap_cic  SaveFormat=Timeseries  SampleTime=-1
      settings: MaxDataPoints=1600001
  tap_fir : ToWorkspace  VariableName=tap_fir  SaveFormat=Timeseries  SampleTime=-1
      settings: MaxDataPoints=1600001
  tap_iq : ToWorkspace  VariableName=tap_iq  SaveFormat=Timeseries  SampleTime=-1
      settings: MaxDataPoints=1600001
  tap_mixer : ToWorkspace  VariableName=tap_mixer  SaveFormat=Timeseries  SampleTime=-1
      settings: MaxDataPoints=1600001
  Out1 : Outport
  wires:
  In1/1 -> ADC_Output_Hold/1
  ADC_Output_Hold/1 -> Mixer_Input/1
  In2/1 -> Mixer_Input/2
  Mixer_Input/1 -> IQ_Mixer/1
  IQ_Mixer/1 -> Mixer_Clock_Boundary/1
  Mixer_Clock_Boundary/1 -> CIC_Equivalent_Boxcar_1/1, tap_mixer/1, Scope_mixer/1, Spectrum_Sample_mixer/1
  CIC_Equivalent_Boxcar_1/1 -> CIC_Equivalent_Boxcar_2/1
  CIC_Equivalent_Boxcar_2/1 -> CIC_Equivalent_Boxcar_3/1
  CIC_Equivalent_Boxcar_3/1 -> Decimate_To_Control/1
  Decimate_To_Control/1 -> FIR_Compensation/1, tap_cic/1, Scope_cic/1, Spectrum_Sample_cic/1
  FIR_Compensation/1 -> IQ_Fixed_Format/1, tap_fir/1, Scope_fir/1, Spectrum_Sample_fir/1
  IQ_Fixed_Format/1 -> Control_Clock_Boundary/1
  Control_Clock_Boundary/1 -> Digital_Pipeline/1
  Digital_Pipeline/1 -> Out1/1, tap_iq/1, Scope_iq/1, Spectrum_Sample_iq/1
  Spectrum_Sample_mixer/1 -> Spectrum_Channel_mixer/1
  Spectrum_Channel_mixer/1 -> Spectrum_mixer/1
  Spectrum_Sample_cic/1 -> Spectrum_Channel_cic/1
  Spectrum_Channel_cic/1 -> Spectrum_cic/1
  Spectrum_Sample_fir/1 -> Spectrum_Channel_fir/1
  Spectrum_Channel_fir/1 -> Spectrum_fir/1
  Spectrum_Sample_iq/1 -> Spectrum_Channel_iq/1
  Spectrum_Channel_iq/1 -> Spectrum_iq/1
  Measured_Clock/1 -> Mixer_Input/3

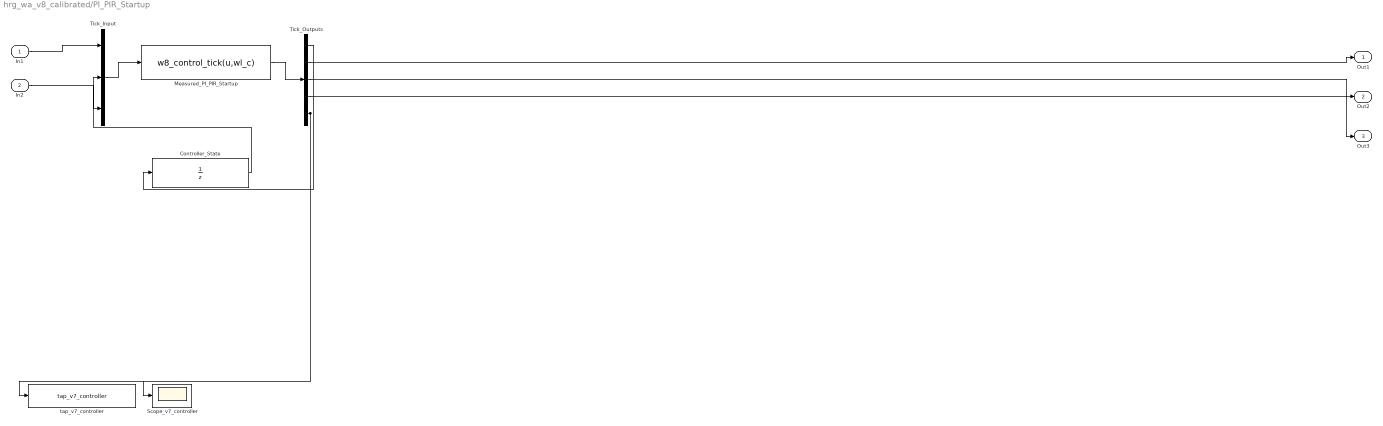
== system hrg_wa_v8_calibrated/PI_PIR_Startup ==
  In1 : Inport
  In2 : Inport  Port=2
  Controller_State : UnitDelay  InitialCondition=zeros(17,1)  SampleTime=wl_Tc  HasFrameUpgradeWarning=on
  Measured_PI_PIR_Startup : MATLABFcn  MATLABFcn=w8_control_tick(u,wl_c)  OutputDimensions=33
  Scope_v7_controller : Scope
  Tick_Input : Mux  Inputs=3
  Tick_Outputs : Demux  Outputs=[17 4 1 3 8]
  tap_v7_controller : ToWorkspace  VariableName=tap_v7_controller  SaveFormat=Timeseries  SampleTime=-1
      settings: MaxDataPoints=1600001
  Out1 : Outport
  Out2 : Outport  Port=2
  Out3 : Outport  Port=3
  wires:
  In1/1 -> Tick_Input/1
  Controller_State/1 -> Tick_Input/2
  In2/1 -> Tick_Input/3
  Tick_Input/1 -> Measured_PI_PIR_Startup/1
  Measured_PI_PIR_Startup/1 -> Tick_Outputs/1
  Tick_Outputs/1 -> Controller_State/1
  Tick_Outputs/2 -> Out1/1
  Tick_Outputs/3 -> Out2/1
  Tick_Outputs/4 -> Out3/1
  Tick_Outputs/5 -> tap_v7_controller/1, Scope_v7_controller/1
